simulink model "rfsoc4x2_ospfb_128"  (R2021a)
settings: Solver=VariableStepAuto  StartTime=0.0  StopTime=2048  RelTol=1e-3
undefined symbols (not defined in the file): pfb_coeff_gen_calc
libraries: xbsIndex_r4 x25898, casper_library_delays x113, casper_library_misc x68, xps_library x1
(part 1 of 221)
settings Model: Creator=leeke  LastModifiedBy=leeke

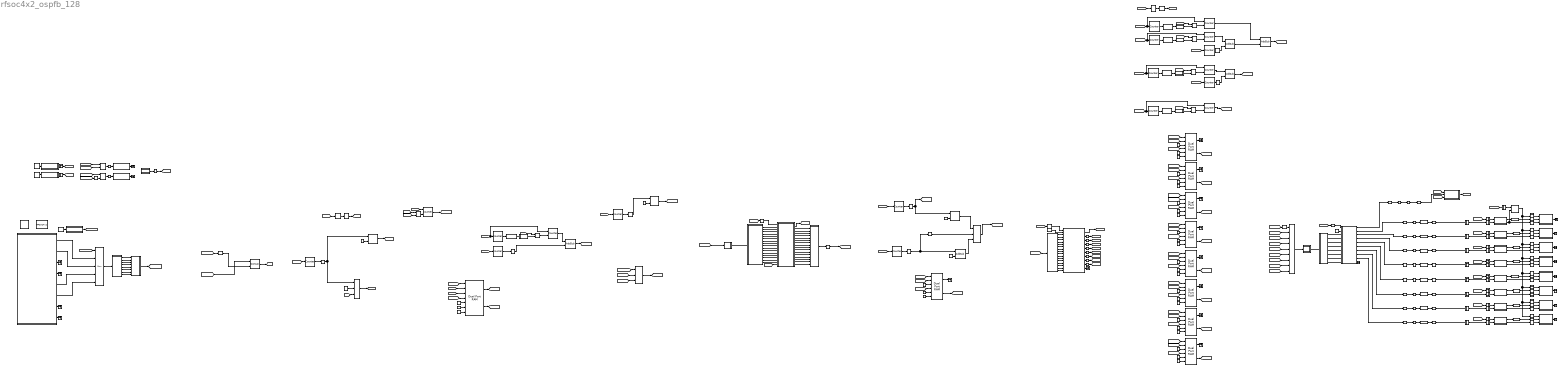
== system rfsoc4x2_ospfb_128 ==
  note: 2nd-stage channelizaton FFT
  note: Coner turn
  note: 1st-stage channelizaton OSPFB
  note: 2x Oversampled polyphase fiter banks
  note: 1st-stage channelizaton OSPFB > Corner Turn > 2nd-stage channelizaton FFT > output
  note: acc_cntrl has a clock
      | cycle latency in generating
      | new_acc signal.
      | Compensate by delaying
      | data here.
  note: 1delay RW mode
  " System Generator" : xbsIndex_r4/ System Generator  Tag=genX  xilinxfamily=zynquplusRFSOC  part=xczu48dr  speed=-2-e  package=ffvg1517  synthesis_tool=XST  clock_wrapper=Clock Enables  directory=/home/leeke/rfsoc4x2/leeke/project/burst/ospfb/2x/8/PFB_FFT/rfsoc4x2_ospfb_128/sysgen  proj_type=Vivado  Synth_file=Vivado Synthesis Defaults  Impl_file=Vivado Implementation Defaults  testbench=off  simulink_period=1  sysclk_period=5  dcm_input_clock_period=10  incr_netlist=off  trim_vbits=Everywhere in SubSystem  dbl_ovrd=According to Block Masks  core_generation=According to Block Masks  run_coregen=off  deprecated_control=off  eval_field=0  block_type=sysgen
  AddSub : xbsIndex_r4/AddSub  mode=Addition  use_carryin=off  use_carryout=off  en=off  latency=0  precision=User Defined  arith_type=Unsigned  n_bits=6-1  bin_pt=0  quantization=Truncate  overflow=Wrap  use_behavioral_HDL=off  hw_selection=Fabric  pipelined=off  dbl_ovrd=off  block_type=addsub
  AddSub1 : xbsIndex_r4/AddSub  mode=Addition  use_carryin=off  use_carryout=off  en=off  latency=0  precision=User Defined  arith_type=Unsigned  n_bits=15-1  bin_pt=0  quantization=Truncate  overflow=Wrap  use_behavioral_HDL=off  hw_selection=Fabric  pipelined=off  dbl_ovrd=off  block_type=addsub
  AddSub2 : xbsIndex_r4/AddSub  mode=Addition  use_carryin=off  use_carryout=off  en=off  latency=0  precision=User Defined  arith_type=Unsigned  n_bits=15-1  bin_pt=0  quantization=Truncate  overflow=Wrap  use_behavioral_HDL=off  hw_selection=Fabric  pipelined=off  dbl_ovrd=off  block_type=addsub
  AddSub3 : xbsIndex_r4/AddSub  mode=Addition  use_carryin=off  use_carryout=off  en=off  latency=0  precision=User Defined  arith_type=Unsigned  n_bits=11  bin_pt=0  quantization=Truncate  overflow=Wrap  use_behavioral_HDL=off  hw_selection=Fabric  pipelined=off  dbl_ovrd=off  block_type=addsub
  AddSub55 : xbsIndex_r4/AddSub  mode=Addition  use_carryin=off  use_carryout=off  en=off  latency=0  precision=User Defined  arith_type=Unsigned  n_bits=5-1  bin_pt=0  quantization=Truncate  overflow=Wrap  use_behavioral_HDL=off  hw_selection=Fabric  pipelined=off  dbl_ovrd=off  block_type=addsub
  Concat6 : xbsIndex_r4/Concat  num_inputs=2  dbl_ovrd=off  block_type=concat
  Constant : Constant  Value=0
  Constant1 : xbsIndex_r4/Constant  const=(2^8)-1  gui_display_data_type=Fixed-point  arith_type=Unsigned  n_bits=8  bin_pt=0  preci_type=Single  exp_width=8  frac_width=24  explicit_period=on  period=1  equ=P=C  opselect=C  inp2=PCIN>>17  opr=+  inp1=P  carry=CIN  dbl_ovrd=off  block_type=constant
  Constant{8..11,16,28,38,43,48} (9 alike) : xbsIndex_r4/Constant  const=1.0  gui_display_data_type=Boolean  arith_type=Boolean  n_bits=1  bin_pt=0  preci_type=Single  exp_width=8  frac_width=24  explicit_period=off  period=1  equ=P=C  opselect=C  inp2=PCIN>>17  opr=+  inp1=P  carry=CIN  dbl_ovrd=off  block_type=constant
  Constant109 : xbsIndex_r4/Constant  const=0  gui_display_data_type=Fixed-point  arith_type=Unsigned  n_bits=64  bin_pt=0  preci_type=Single  exp_width=8  frac_width=24  explicit_period=off  period=1  equ=P=C  opselect=C  inp2=PCIN>>17  opr=+  inp1=P  carry=CIN  dbl_ovrd=off  block_type=constant
  Constant110 : xbsIndex_r4/Constant  const=0  gui_display_data_type=Fixed-point  arith_type=Unsigned  n_bits=16 * 16  bin_pt=0  preci_type=Single  exp_width=8  frac_width=24  explicit_period=off  period=1  equ=P=C  opselect=C  inp2=PCIN>>17  opr=+  inp1=P  carry=CIN  dbl_ovrd=off  block_type=constant
  Constant{17,19,30,37,40,42,45,47,50,111} (10 alike) : xbsIndex_r4/Constant  const=0  gui_display_data_type=Boolean  arith_type=Boolean  n_bits=144  bin_pt=0  preci_type=Single  exp_width=8  frac_width=24  explicit_period=off  period=1  equ=P=C  opselect=C  inp2=PCIN>>17  opr=+  inp1=P  carry=CIN  dbl_ovrd=off  block_type=constant
  Constant112 : xbsIndex_r4/Constant  const=1  gui_display_data_type=Boolean  arith_type=Boolean  n_bits=144  bin_pt=0  preci_type=Single  exp_width=8  frac_width=24  explicit_period=off  period=1  equ=P=C  opselect=C  inp2=PCIN>>17  opr=+  inp1=P  carry=CIN  dbl_ovrd=off  block_type=constant
  Constant113 : xbsIndex_r4/Constant  const=0  gui_display_data_type=Fixed-point  arith_type=Unsigned  n_bits=1  bin_pt=0  preci_type=Single  exp_width=8  frac_width=24  explicit_period=off  period=1  equ=P=C  opselect=C  inp2=PCIN>>17  opr=+  inp1=P  carry=CIN  dbl_ovrd=off  block_type=constant
  Constant114 : xbsIndex_r4/Constant  const=(2^8 / 2^4) - 1  gui_display_data_type=Fixed-point  arith_type=Unsigned  n_bits=log2((2^8 / 2^4))  bin_pt=0  preci_type=Single  exp_width=8  frac_width=24  explicit_period=off  period=1  equ=P=C  opselect=C  inp2=PCIN>>17  opr=+  inp1=P  carry=CIN  dbl_ovrd=off  block_type=constant
  Constant{12..13,18,29,39,41,44,46,49} (9 alike) : xbsIndex_r4/Constant  const=0  gui_display_data_type=Fixed-point  arith_type=Unsigned  n_bits=144*2  bin_pt=0  preci_type=Single  exp_width=8  frac_width=24  explicit_period=off  period=1  equ=P=C  opselect=C  inp2=PCIN>>17  opr=+  inp1=P  carry=CIN  dbl_ovrd=off  block_type=constant
  Constant2 : Constant  Value=0
  Constant20 : xbsIndex_r4/Constant  const=32/2  gui_display_data_type=Fixed-point  arith_type=Unsigned  n_bits=6-1  bin_pt=0  preci_type=Single  exp_width=8  frac_width=24  explicit_period=off  period=1  equ=P=C  opselect=C  inp2=PCIN>>17  opr=+  inp1=P  carry=CIN  dbl_ovrd=off  block_type=constant
  Constant21 : xbsIndex_r4/Constant  const=32/2  gui_display_data_type=Fixed-point  arith_type=Unsigned  n_bits=6-1  bin_pt=0  preci_type=Single  exp_width=8  frac_width=24  explicit_period=off  period=1  equ=P=C  opselect=C  inp2=PCIN>>17  opr=+  inp1=P  carry=CIN  dbl_ovrd=off  block_type=constant
  Constant3 : Constant  Value=2
  Constant51 : xbsIndex_r4/Constant  const=(2^9)-1  gui_display_data_type=Fixed-point  arith_type=Unsigned  n_bits=9  bin_pt=0  preci_type=Single  exp_width=8  frac_width=24  explicit_period=on  period=1  equ=P=C  opselect=C  inp2=PCIN>>17  opr=+  inp1=P  carry=CIN  dbl_ovrd=off  block_type=constant
  Convert2 : xbsIndex_r4/Convert  gui_display_data_type=Boolean  arith_type=Boolean  n_bits=16  bin_pt=14  float_type=Single  exp_bits=8  fraction_bits=24  quantization=Truncate  overflow=Wrap  en=off  latency=1  pipeline=off  dbl_ovrd=off  block_type=convert
  Convert6 : xbsIndex_r4/Convert  gui_display_data_type=Boolean  arith_type=Boolean  n_bits=16  bin_pt=14  float_type=Single  exp_bits=8  fraction_bits=24  quantization=Truncate  overflow=Wrap  en=off  latency=1  pipeline=off  dbl_ovrd=off  block_type=convert
  Counter1 : xbsIndex_r4/Counter  cnt_type=Count Limited  cnt_to=(16384/2)-512  operation=Up  start_count=0  cnt_by_val=512  arith_type=Unsigned  n_bits=14-1  bin_pt=0  load_pin=off  rst=on  en=off  explicit_period=on  period=1  use_behavioral_HDL=off  implementation=Fabric  dbl_ovrd=off  block_type=counter
  Counter13 : xbsIndex_r4/Counter  cnt_type=Free Running  cnt_to=1023  operation=Up  start_count=16/2  cnt_by_val=1  arith_type=Unsigned  n_bits=5-1  bin_pt=0  load_pin=off  rst=on  en=off  explicit_period=on  period=1  use_behavioral_HDL=off  implementation=Fabric  dbl_ovrd=off  block_type=counter
  Counter14 : xbsIndex_r4/Counter  cnt_type=Free Running  cnt_to=Inf  operation=Up  start_count=0  cnt_by_val=1  arith_type=Unsigned  n_bits=7-1  bin_pt=0  load_pin=off  rst=on  en=off  explicit_period=on  period=1  use_behavioral_HDL=off  implementation=Fabric  dbl_ovrd=off  block_type=counter
  Counter15 : xbsIndex_r4/Counter  cnt_type=Free Running  cnt_to=1023  operation=Up  start_count=0  cnt_by_val=1  arith_type=Unsigned  n_bits=6-1  bin_pt=0  load_pin=off  rst=on  en=off  explicit_period=on  period=1  use_behavioral_HDL=off  implementation=Fabric  dbl_ovrd=off  block_type=counter
  Counter16 : xbsIndex_r4/Counter  cnt_type=Free Running  cnt_to=Inf  operation=Up  start_count=0  cnt_by_val=1  arith_type=Unsigned  n_bits=7-1  bin_pt=0  load_pin=off  rst=on  en=off  explicit_period=on  period=1  use_behavioral_HDL=off  implementation=Fabric  dbl_ovrd=off  block_type=counter
  Counter17 : xbsIndex_r4/Counter  cnt_type=Free Running  cnt_to=16  operation=Up  start_count=1024  cnt_by_val=128/2  arith_type=Unsigned  n_bits=11  bin_pt=0  load_pin=off  rst=on  en=on  explicit_period=on  period=1  use_behavioral_HDL=off  implementation=Fabric  dbl_ovrd=off  block_type=counter
  Counter18 : xbsIndex_r4/Counter  cnt_type=Free Running  cnt_to=Inf  operation=Up  start_count=0  cnt_by_val=1  arith_type=Unsigned  n_bits=9  bin_pt=0  load_pin=off  rst=on  en=off  explicit_period=on  period=1  use_behavioral_HDL=off  implementation=Fabric  dbl_ovrd=off  block_type=counter
  Counter19 : xbsIndex_r4/Counter  cnt_type=Free Running  cnt_to=Inf  operation=Up  start_count=0  cnt_by_val=1  arith_type=Unsigned  n_bits=1  bin_pt=0  load_pin=off  rst=off  en=on  explicit_period=on  period=1  use_behavioral_HDL=off  implementation=Fabric  dbl_ovrd=off  block_type=counter
  Counter2 : xbsIndex_r4/Counter  cnt_type=Free Running  cnt_to=0  operation=Up  start_count=0  cnt_by_val=1  arith_type=Unsigned  n_bits=9  bin_pt=0  load_pin=off  rst=on  en=on  explicit_period=on  period=1  use_behavioral_HDL=off  implementation=Fabric  dbl_ovrd=off  block_type=counter
  Counter3 : xbsIndex_r4/Counter  cnt_type=Free Running  cnt_to=0  operation=Up  start_count=0  cnt_by_val=16384/2  arith_type=Unsigned  n_bits=15-1  bin_pt=0  load_pin=off  rst=on  en=on  explicit_period=on  period=1  use_behavioral_HDL=off  implementation=Fabric  dbl_ovrd=off  block_type=counter
  Counter4 : xbsIndex_r4/Counter  cnt_type=Free Running  cnt_to=Inf  operation=Up  start_count=0  cnt_by_val=1  arith_type=Unsigned  n_bits=14-1  bin_pt=0  load_pin=off  rst=on  en=off  explicit_period=on  period=1  use_behavioral_HDL=off  implementation=Fabric  dbl_ovrd=off  block_type=counter
  Counter55 : xbsIndex_r4/Counter  cnt_type=Free Running  cnt_to=1023  operation=Up  start_count=0  cnt_by_val=1  arith_type=Unsigned  n_bits=1  bin_pt=0  load_pin=off  rst=on  en=off  explicit_period=on  period=1  use_behavioral_HDL=off  implementation=Fabric  dbl_ovrd=off  block_type=counter
  Counter56 : xbsIndex_r4/Counter  cnt_type=Free Running  cnt_to=1023  operation=Up  start_count=0  cnt_by_val=1  arith_type=Unsigned  n_bits=log2((2^8 / 2^4))  bin_pt=0  load_pin=off  rst=on  en=on  explicit_period=on  period=1  use_behavioral_HDL=off  implementation=Fabric  dbl_ovrd=off  block_type=counter
  Counter57 : xbsIndex_r4/Counter  cnt_type=Free Running  cnt_to=Inf  operation=Up  start_count=0  cnt_by_val=1  arith_type=Unsigned  n_bits=1  bin_pt=0  load_pin=off  rst=off  en=on  explicit_period=on  period=1  use_behavioral_HDL=off  implementation=Fabric  dbl_ovrd=off  block_type=counter
  Counter58 : xbsIndex_r4/Counter  cnt_type=Free Running  cnt_to=0  operation=Up  start_count=8  cnt_by_val=16/2  arith_type=Unsigned  n_bits=5-1  bin_pt=0  load_pin=off  rst=on  en=on  explicit_period=on  period=1  use_behavioral_HDL=off  implementation=Fabric  dbl_ovrd=off  block_type=counter
  Counter59 : xbsIndex_r4/Counter  cnt_type=Free Running  cnt_to=Inf  operation=Up  start_count=16/2  cnt_by_val=1  arith_type=Unsigned  n_bits=5-1  bin_pt=0  load_pin=off  rst=on  en=off  explicit_period=on  period=1  use_behavioral_HDL=off  implementation=Fabric  dbl_ovrd=off  block_type=counter
  Counter6 : xbsIndex_r4/Counter  cnt_type=Free Running  cnt_to=Inf  operation=Up  start_count=0  cnt_by_val=1  arith_type=Unsigned  n_bits=5-1  bin_pt=0  load_pin=off  rst=on  en=off  explicit_period=on  period=1  use_behavioral_HDL=off  implementation=Fabric  dbl_ovrd=off  block_type=counter
  Counter60 : xbsIndex_r4/Counter  cnt_type=Free Running  cnt_to=1023  operation=Up  start_count=0  cnt_by_val=1  arith_type=Unsigned  n_bits=4-1  bin_pt=0  load_pin=off  rst=on  en=off  explicit_period=on  period=1  use_behavioral_HDL=off  implementation=Fabric  dbl_ovrd=off  block_type=counter
  Counter61 : xbsIndex_r4/Counter  cnt_type=Free Running  cnt_to=1023  operation=Up  start_count=0  cnt_by_val=1  arith_type=Unsigned  n_bits=log2((2^8 / 2^4))  bin_pt=0  load_pin=off  rst=on  en=off  explicit_period=on  period=1  use_behavioral_HDL=off  implementation=Fabric  dbl_ovrd=off  block_type=counter
  Counter7 : xbsIndex_r4/Counter  cnt_type=Free Running  cnt_to=16  operation=Up  start_count=0  cnt_by_val=1  arith_type=Unsigned  n_bits=2+1  bin_pt=0  load_pin=off  rst=on  en=on  explicit_period=on  period=1  use_behavioral_HDL=off  implementation=Fabric  dbl_ovrd=off  block_type=counter
  Delay{1..4,49..50,57..58,62,66,68..71,74..75,77..78,81,83..87,89..90} (26 alike) : xbsIndex_r4/Delay  rst=off  infoeditControl=Selection of Reset will increase slice count due to use of real FFs and instead of SRLs  en=off  latency=1  reg_retiming=on  dbl_ovrd=off  block_type=delay
  Delay{13..14,17,23,59..61,136..139} (11 alike) : xbsIndex_r4/Delay  rst=off  infoeditControl=Selection of Reset will increase slice count due to use of real FFs and instead of SRLs  en=off  latency=1  reg_retiming=off  dbl_ovrd=off  block_type=delay
  Delay15 : xbsIndex_r4/Delay  rst=off  infoeditControl=Selection of Reset will increase slice count due to use of real FFs and instead of SRLs  en=off  latency=16/2  reg_retiming=off  dbl_ovrd=off  block_type=delay
  Delay16 : xbsIndex_r4/Delay  rst=off  infoeditControl=Selection of Reset will increase slice count due to use of real FFs and instead of SRLs  en=off  latency=2  reg_retiming=off  dbl_ovrd=off  block_type=delay
  Delay{6,21,33,63..65,67,72,76,79..80,82,88} (13 alike) : xbsIndex_r4/Delay  rst=off  infoeditControl=Selection of Reset will increase slice count due to use of real FFs and instead of SRLs  en=off  latency=2  reg_retiming=on  dbl_ovrd=off  block_type=delay
  Delay73 : xbsIndex_r4/Delay  rst=off  infoeditControl=Selection of Reset will increase slice count due to use of real FFs and instead of SRLs  en=off  latency=5  reg_retiming=on  dbl_ovrd=off  block_type=delay
  Dual Port RAM{1..4,11..14} (8 alike) : xbsIndex_r4/Dual Port RAM  depth=16384  initVector=0  distributed_mem=Block RAM  init_a=0  init_b=0  rst_a=off  rst_b=off  en_a=off  en_b=off  latency=1  write_mode_A=Read Before Write  write_mode_B=Read Before Write  optimize=Area  dbl_ovrd=off  simulation_type=fast_sim  block_type=dpram
  Dual Port RAM16 : xbsIndex_r4/Dual Port RAM  depth=(2^8) / (2^4)  initVector=0  distributed_mem=Block RAM  init_a=0  init_b=0  rst_a=off  rst_b=off  en_a=off  en_b=on  latency=1  write_mode_A=Read After Write  write_mode_B=Read Before Write  optimize=Area  dbl_ovrd=off  simulation_type=fast_sim  block_type=dpram
  Dual Port RAM6 : xbsIndex_r4/Dual Port RAM  depth=32  initVector=0  distributed_mem=Block RAM  init_a=0  init_b=0  rst_a=off  rst_b=off  en_a=off  en_b=off  latency=1  write_mode_A=Read Before Write  write_mode_B=Read Before Write  optimize=Area  dbl_ovrd=off  simulation_type=fast_sim  block_type=dpram
  Logical{2..3,9..10,12..13} (6 alike) : xbsIndex_r4/Logical  logical_function=AND  inputs=2  en=off  latency=0  precision=Full  arith_type=Unsigned  n_bits=16  bin_pt=0  align_bp=on  dbl_ovrd=off  block_type=logical
  Mux : xbsIndex_r4/Mux  inputs=4  en=off  latency=2  precision=Full  arith_type=Unsigned  n_bits=16  bin_pt=14  quantization=Truncate  overflow=Wrap  dbl_ovrd=off  block_type=mux
  Mux13 : xbsIndex_r4/Mux  inputs=2  en=off  latency=0  precision=Full  arith_type=Unsigned  n_bits=16  bin_pt=14  quantization=Truncate  overflow=Wrap  dbl_ovrd=off  block_type=mux
  Mux14 : xbsIndex_r4/Mux  inputs=2  en=off  latency=0  precision=Full  arith_type=Unsigned  n_bits=16  bin_pt=14  quantization=Truncate  overflow=Wrap  dbl_ovrd=off  block_type=mux
  Mux3 : xbsIndex_r4/Mux  inputs=2  en=off  latency=0  precision=Full  arith_type=Unsigned  n_bits=16  bin_pt=14  quantization=Truncate  overflow=Wrap  dbl_ovrd=off  block_type=mux
  Mux5 : xbsIndex_r4/Mux  inputs=8  en=off  latency=0  precision=Full  arith_type=Unsigned  n_bits=16  bin_pt=14  quantization=Truncate  overflow=Wrap  dbl_ovrd=off  block_type=mux
  RFSoC4x2 : xps_library/Platforms/RFSoC4x2  Tag=xps:xsg  hw_sys=rfsoc4x2:xczu48dr  clk_src=adc_clk  clk_rate=200  pl_clk_rate=100  sample_period=1  synthesis_tool=XST
      settings: SourceProductName=CASPER XPS Blockset
  Reinterpret{7,10..16} (8 alike) : xbsIndex_r4/Reinterpret  force_arith_type=on  arith_type=Unsigned  force_bin_pt=on  bin_pt=0  block_type=reinterpret
      settings: infoedit="Changes signal type without altering the binary representation.   You can changed the signal between signed and unsigned, and relocate the binary point.<P><P>Hardware notes: In hardware this block costs nothing.<P><P>Example:  Suppose the input is 6 bits wide, signed, with 2 fractional bits, and the output is forced to unsigned with 0 fractional bits.  Then an input of -2.0 (1110.00 in binary 2's complement) becomes an output of 56 (111000 in binary)."  block_version=10.1.3
  Relational : xbsIndex_r4/Relational  mode=a<b  op_type=Bool  en=off  latency=0  dbl_ovrd=off  block_type=relational
  Relational2 : xbsIndex_r4/Relational  mode=a>b  op_type=Bool  en=off  latency=0  dbl_ovrd=off  block_type=relational
  Relational3 : xbsIndex_r4/Relational  mode=a<b  op_type=Bool  en=off  latency=1  dbl_ovrd=off  block_type=relational
  Slice{1,3..5,14} (5 alike) : xbsIndex_r4/Slice  nbits=1  boolean_output=on  mode=Upper Bit Location + Width  bit1=0  base1=MSB of Input  bit0=0  base0=LSB of Input  dbl_ovrd=off  block_type=slice
  Terminator{1..4,6..7,11,16,18..23,25..34,38} (25 alike) : Terminator
  acc_cnt : Subsystem  Tag=xps:sw_reg  AncestorBlock=xps_library/Memory/software_register  mask(swreg){io_dir=To Processor, io_delay=0, init_val=0, sample_period=1, names=reg, bitwidths=32, bin_pts=0, arith_types=0, sim_port=on, show_format=off}
      mask prompts: io_dir "I/O direction"; io_delay "I/O delay"; init_val "Initial Value"; sample_period "Sample period"; names "Bitfield names [msb...lsb]"; bitwidths "Bitfield widths"; bin_pts "Bitfield binary pts"; arith_types "Bitfield types, ufix=0, fix=1, bool=2"; sim_port "Provide sim input/output?"; show_format "Print format string?"
      mask help: A 32-bit software-accessible register. Can be divided into bitfields of varying widths and types using the fields in the block mask.
      mask init:
      | swreg_init(gcb)
      settings: AttributesFormatString=1output
      mask TypeOptions io_dir: To Processor | From Processor
      mask Callback io_dir:
      | mask_enables = get_param(gcb, 'MaskEnables');
      | mask_names = get_param(gcb, 'MaskNames');
      | if strcmp(get_param(gcb, 'io_dir'), 'To Processor'),
      |     mask_enables{ismember(mask_names, 'sample_period')} = 'off';
      | else
      |     mask_enables{ismember(mask_names, 'sample_period')} = 'on';
      | end
      | set_param(gcb, 'MaskEnables', mask_enables);
      mask DialogControl ParameterTabVar0 Prompt: Setup
  acc_cntr : xbsIndex_r4/Counter  cnt_type=Free Running  cnt_to=Inf  operation=Up  start_count=0  cnt_by_val=1  arith_type=Unsigned  n_bits=32  bin_pt=0  load_pin=off  rst=on  en=on  explicit_period=on  period=1  use_behavioral_HDL=off  implementation=Fabric  use_rpm=off  dbl_ovrd=off  block_type=counter
  acc_cntrl2 : Subsystem  mask{chan_bits=13}
      mask prompts: chan_bits "Number of Channels (2^?)"
  acc_len : Subsystem  Tag=xps:sw_reg  AncestorBlock=xps_library/Memory/software_register  mask(swreg){io_dir=From Processor, io_delay=0, init_val=0, sample_period=1, names=reg, bitwidths=32, bin_pts=0, arith_types=0, sim_port=on, show_format=off}
      mask prompts: io_dir "I/O direction"; io_delay "I/O delay"; init_val "Initial Value"; sample_period "Sample period"; names "Bitfield names [msb...lsb]"; bitwidths "Bitfield widths"; bin_pts "Bitfield binary pts"; arith_types "Bitfield types, ufix=0, fix=1, bool=2"; sim_port "Provide sim input/output?"; show_format "Print format string?"
      mask help: A 32-bit software-accessible register. Can be divided into bitfields of varying widths and types using the fields in the block mask.
      mask init:
      | swreg_init(gcb)
      settings: AttributesFormatString=1input
      mask TypeOptions io_dir: To Processor | From Processor
      mask Callback io_dir:
      | mask_enables = get_param(gcb, 'MaskEnables');
      | mask_names = get_param(gcb, 'MaskNames');
      | if strcmp(get_param(gcb, 'io_dir'), 'To Processor'),
      |     mask_enables{ismember(mask_names, 'sample_period')} = 'off';
      | else
      |     mask_enables{ismember(mask_names, 'sample_period')} = 'on';
      | end
      | set_param(gcb, 'MaskEnables', mask_enables);
      mask DialogControl ParameterTabVar0 Prompt: Setup
  adc_chan_sel : Subsystem  Tag=xps:sw_reg  AncestorBlock=xps_library/Memory/software_register  mask(swreg){io_dir=From Processor, io_delay=0, init_val=dec2hex(0), sample_period=1, names=reg, bitwidths=2, bin_pts=0, arith_types=0, sim_port=on, show_format=on}
      mask prompts: io_dir "I/O direction"; io_delay "I/O delay"; init_val "Initial Value"; sample_period "Sample period"; names "Bitfield names [msb...lsb]"; bitwidths "Bitfield widths"; bin_pts "Bitfield binary pts"; arith_types "Bitfield types, ufix=0, fix=1, bool=2"; sim_port "Provide sim input/output?"; show_format "Print format string?"
      mask help: A 32-bit software-accessible register. Can be divided into bitfields of varying widths and types using the fields in the block mask.
      mask init:
      | swreg_init(gcb)
      settings: AttributesFormatString=1input:uf2.0 = 2 bits
      mask TypeOptions io_dir: To Processor | From Processor
      mask Callback io_dir:
      | mask_enables = get_param(gcb, 'MaskEnables');
      | mask_names = get_param(gcb, 'MaskNames');
      | if strcmp(get_param(gcb, 'io_dir'), 'To Processor'),
      |     mask_enables{ismember(mask_names, 'sample_period')} = 'off';
      | else
      |     mask_enables{ismember(mask_names, 'sample_period')} = 'on';
      | end
      | set_param(gcb, 'MaskEnables', mask_enables);
      mask DialogControl ParameterTabVar0 Prompt: Setup
  bus_create : Subsystem  AncestorBlock=casper_library_flow_control/bus_create  mask(bus_create){inputNum=8}
      mask prompts: inputNum "Number of inputs:"
      mask init:
      | bus_create_init(gcb,...
      |     'inputNum', inputNum);
  bus_create2 : Subsystem  AncestorBlock=casper_library_flow_control/bus_create  mask(bus_create){inputNum=16}
      mask prompts: inputNum "Number of inputs:"
      mask init:
      | bus_create_init(gcb,...
      |     'inputNum', inputNum);
  bus_expand : Subsystem  AncestorBlock=casper_library_flow_control/bus_expand  mask(bus_expand){mode=divisions of equal size, outputNum=16, outputWidth=16, outputBinaryPt=0, outputArithmeticType=0, show_format=off, outputToWorkspace=off, variablePrefix=out, outputToModelAsWell=on}
      mask prompts: outputNum "Number of outputs:"; outputWidth "Output width:"; outputBinaryPt "Output binary point position:"; outputArithmeticType "Output arithmetic type (ufix=0, fix=1, bool=2):"; show_format "Print format string?"; outputToWorkspace "Output to workspace?"; variablePrefix "Variable name prefix:"; outputToModelAsWell "Output to model as well?"
      mask help:
      | Expands a 'bus' made using a bus_create or Xilinx
      | concat block.
      | The input will be divided into the specified number
      | of outputs with the specified arithmetic types.
      | Divisions are made from most significant bit.
      mask init:
      | bus_expand_init(gcb,...
      |     'mode', mode, ...
      |     'outputNum', outputNum, ...
      |     'outputWidth', outputWidth, ...
      |     'outputBinaryPt', outputBinaryPt, ...
      |     'outputArithmeticType', outputArithmeticType, ...
      |     'show_format', show_format, ...
      |     'outputToWorkspace', outputToWorkspace, ...
      |     'variablePrefix', variablePrefix, ...
      |     'outputToModelAsWell', outputToModelAsWell);
      settings: AttributesFormatString=16 outputs
      mask TypeOptions mode: divisions of equal size | divisions of arbitrary size
      mask Callback mode: %bus_expand_callback();
      mask Callback outputWidth: %bus_expand_callback();
      mask Callback outputToWorkspace: %bus_expand_callback();
  bus_expand1 : Subsystem  AncestorBlock=casper_library_flow_control/bus_expand  mask(bus_expand){mode=divisions of equal size, outputNum=8, outputWidth=16, outputBinaryPt=0, outputArithmeticType=0, show_format=off, outputToWorkspace=off, variablePrefix=out, outputToModelAsWell=on}
      mask prompts: outputNum "Number of outputs:"; outputWidth "Output width:"; outputBinaryPt "Output binary point position:"; outputArithmeticType "Output arithmetic type (ufix=0, fix=1, bool=2):"; show_format "Print format string?"; outputToWorkspace "Output to workspace?"; variablePrefix "Variable name prefix:"; outputToModelAsWell "Output to model as well?"
      mask help:
      | Expands a 'bus' made using a bus_create or Xilinx
      | concat block.
      | The input will be divided into the specified number
      | of outputs with the specified arithmetic types.
      | Divisions are made from most significant bit.
      mask init: same as rfsoc4x2_ospfb_128/bus_expand
      settings: AttributesFormatString=8 outputs
      mask TypeOptions mode: divisions of equal size | divisions of arbitrary size
      mask Callback mode: %bus_expand_callback();
      mask Callback outputWidth: %bus_expand_callback();
      mask Callback outputToWorkspace: %bus_expand_callback();
  bus_expand3 : Subsystem  AncestorBlock=casper_library_flow_control/bus_expand  mask(bus_expand){mode=divisions of equal size, outputNum=16, outputWidth=18, outputBinaryPt=17, outputArithmeticType=1, show_format=off, outputToWorkspace=off, variablePrefix=out, outputToModelAsWell=on}
      mask prompts: outputNum "Number of outputs:"; outputWidth "Output width:"; outputBinaryPt "Output binary point position:"; outputArithmeticType "Output arithmetic type (ufix=0, fix=1, bool=2):"; show_format "Print format string?"; outputToWorkspace "Output to workspace?"; variablePrefix "Variable name prefix:"; outputToModelAsWell "Output to model as well?"
      mask help:
      | Expands a 'bus' made using a bus_create or Xilinx
      | concat block.
      | The input will be divided into the specified number
      | of outputs with the specified arithmetic types.
      | Divisions are made from most significant bit.
      mask init: same as rfsoc4x2_ospfb_128/bus_expand
      settings: AttributesFormatString=16 outputs
      mask TypeOptions mode: divisions of equal size | divisions of arbitrary size
      mask Callback mode: %bus_expand_callback();
      mask Callback outputWidth: %bus_expand_callback();
      mask Callback outputToWorkspace: %bus_expand_callback();
  bus_expand4 : Subsystem  AncestorBlock=casper_library_flow_control/bus_expand  mask(bus_expand){mode=divisions of equal size, outputNum=8, outputWidth=36, outputBinaryPt=0, outputArithmeticType=0, show_format=off, outputToWorkspace=off, variablePrefix=out, outputToModelAsWell=on}
      mask prompts: outputNum "Number of outputs:"; outputWidth "Output width:"; outputBinaryPt "Output binary point position:"; outputArithmeticType "Output arithmetic type (ufix=0, fix=1, bool=2):"; show_format "Print format string?"; outputToWorkspace "Output to workspace?"; variablePrefix "Variable name prefix:"; outputToModelAsWell "Output to model as well?"
      mask help:
      | Expands a 'bus' made using a bus_create or Xilinx
      | concat block.
      | The input will be divided into the specified number
      | of outputs with the specified arithmetic types.
      | Divisions are made from most significant bit.
      mask init: same as rfsoc4x2_ospfb_128/bus_expand
      settings: AttributesFormatString=8 outputs
      mask TypeOptions mode: divisions of equal size | divisions of arbitrary size
      mask Callback mode: %bus_expand_callback();
      mask Callback outputWidth: %bus_expand_callback();
      mask Callback outputToWorkspace: %bus_expand_callback();
  cnt_rst : Subsystem  Tag=xps:sw_reg  AncestorBlock=xps_library/Memory/software_register  mask(swreg){io_dir=From Processor, io_delay=0, init_val=dec2hex(0), sample_period=1, names=reg, bitwidths=1, bin_pts=0, arith_types=2, sim_port=on, show_format=on}
      mask prompts: io_dir "I/O direction"; io_delay "I/O delay"; init_val "Initial Value"; sample_period "Sample period"; names "Bitfield names [msb...lsb]"; bitwidths "Bitfield widths"; bin_pts "Bitfield binary pts"; arith_types "Bitfield types, ufix=0, fix=1, bool=2"; sim_port "Provide sim input/output?"; show_format "Print format string?"
      mask help: A 32-bit software-accessible register. Can be divided into bitfields of varying widths and types using the fields in the block mask.
      mask init:
      | swreg_init(gcb)
      settings: AttributesFormatString=1input:b = 1 bits
      mask TypeOptions io_dir: To Processor | From Processor
      mask Callback io_dir:
      | mask_enables = get_param(gcb, 'MaskEnables');
      | mask_names = get_param(gcb, 'MaskNames');
      | if strcmp(get_param(gcb, 'io_dir'), 'To Processor'),
      |     mask_enables{ismember(mask_names, 'sample_period')} = 'off';
      | else
      |     mask_enables{ismember(mask_names, 'sample_period')} = 'on';
      | end
      | set_param(gcb, 'MaskEnables', mask_enables);
      mask DialogControl ParameterTabVar0 Prompt: Setup
  edge_detect1 : Subsystem  AncestorBlock=casper_library_misc/edge_detect  mask(edge_detect){edge=Falling, polarity=Active High, x_in=[0 0.08 0.08 0.16 0.16 0.24 0.24 0.32 0.32 0.4], y_in=[-1 -1  1  1  1  1  1  1  1  1], x_out=[0.6 0.68 0.68 0.76 0.76 0.84 0.84 0.92 0.92 1], y_out=[-1 -1  1  1 -1 -1 -1 -1 -1 -1]}
      mask prompts: edge "Edge Type"; polarity "Output Polarity"; x_in "Input X Positions"; y_in "Input Y Positions"; x_out "Output X Positions"; y_out "Output Y Positions"
      mask help: Output is active for one-cycle after each edge of the specified type (i.e. rising, falling or both).
      mask init:
      | edge_detect_init(gcb,...
      |     'edge',edge,...
      |     'polarity',polarity,...
      |     'x_in',x_in,...
      |     'x_out',x_out,...
      |     'y_in',y_in,...
      |     'y_out',y_out);
      | 
      | x_in_num=str2num(getfield(getfield(get_param(gcb,'UserData'),'parameters'),'x_in'));
      | x_out_num=str2num(getfield(getfield(get_param(gcb,'UserData'),'parameters'),'x_out'));
      | y_in_num=str2num(getfield(getfield(get_param(gcb,'UserData'),'parameters'),'y_in'));
      | y_out_num=str2num(getfield(getfield(get_param(gcb,'UserData'),'parameters'),'y_out'));
      settings: AttributesFormatString=|
      | falling edges
      | active high
      mask Help: Output is active for one-cycle after each edge of the specified type (i.e. rising, falling, or both).  Latency is zero.
      mask TypeOptions edge: Rising | Falling | Both
      mask TypeOptions polarity: Active High | Active Low
      mask Display:
      | plot(x_in_num,0.5+y_in_num*0.2);
      | plot(x_out_num,0.5+y_out_num*0.2);
  edge_detect15 : Subsystem  AncestorBlock=casper_library_misc/edge_detect  mask(edge_detect){edge=Falling, polarity=Active High, x_in=[0 0.08 0.08 0.16 0.16 0.24 0.24 0.32 0.32 0.4], y_in=[-1 -1  1  1  1  1  1  1  1  1], x_out=[0.6 0.68 0.68 0.76 0.76 0.84 0.84 0.92 0.92 1], y_out=[-1 -1  1  1 -1 -1 -1 -1 -1 -1]}
      mask prompts: edge "Edge Type"; polarity "Output Polarity"; x_in "Input X Positions"; y_in "Input Y Positions"; x_out "Output X Positions"; y_out "Output Y Positions"
      mask help: Output is active for one-cycle after each edge of the specified type (i.e. rising, falling or both).
      mask init: same as rfsoc4x2_ospfb_128/edge_detect1
      settings: AttributesFormatString=|
      | falling edges
      | active high
      mask Help: Output is active for one-cycle after each edge of the specified type (i.e. rising, falling, or both).  Latency is zero.
      mask TypeOptions edge: Rising | Falling | Both
      mask TypeOptions polarity: Active High | Active Low
      mask Display:
      | plot(x_in_num,0.5+y_in_num*0.2);
      | plot(x_out_num,0.5+y_out_num*0.2);
  edge_detect2 : Subsystem  AncestorBlock=casper_library_misc/edge_detect  mask(edge_detect){edge=Falling, polarity=Active High, x_in=[0 0.08 0.08 0.16 0.16 0.24 0.24 0.32 0.32 0.4], y_in=[-1 -1  1  1  1  1  1  1  1  1], x_out=[0.6 0.68 0.68 0.76 0.76 0.84 0.84 0.92 0.92 1], y_out=[-1 -1  1  1 -1 -1 -1 -1 -1 -1]}
      mask prompts: edge "Edge Type"; polarity "Output Polarity"; x_in "Input X Positions"; y_in "Input Y Positions"; x_out "Output X Positions"; y_out "Output Y Positions"
      mask help: Output is active for one-cycle after each edge of the specified type (i.e. rising, falling or both).
      mask init: same as rfsoc4x2_ospfb_128/edge_detect1
      settings: AttributesFormatString=|
      | falling edges
      | active high
      mask Help: Output is active for one-cycle after each edge of the specified type (i.e. rising, falling, or both).  Latency is zero.
      mask TypeOptions edge: Rising | Falling | Both
      mask TypeOptions polarity: Active High | Active Low
      mask Display:
      | plot(x_in_num,0.5+y_in_num*0.2);
      | plot(x_out_num,0.5+y_out_num*0.2);
  edge_detect3 : Subsystem  AncestorBlock=casper_library_misc/edge_detect  mask(edge_detect){edge=Falling, polarity=Active High, x_in=[0 0.08 0.08 0.16 0.16 0.24 0.24 0.32 0.32 0.4], y_in=[-1 -1  1  1  1  1  1  1  1  1], x_out=[0.6 0.68 0.68 0.76 0.76 0.84 0.84 0.92 0.92 1], y_out=[-1 -1  1  1 -1 -1 -1 -1 -1 -1]}
      mask prompts: edge "Edge Type"; polarity "Output Polarity"; x_in "Input X Positions"; y_in "Input Y Positions"; x_out "Output X Positions"; y_out "Output Y Positions"
      mask help: Output is active for one-cycle after each edge of the specified type (i.e. rising, falling or both).
      mask init: same as rfsoc4x2_ospfb_128/edge_detect1
      settings: AttributesFormatString=|
      | falling edges
      | active high
      mask Help: Output is active for one-cycle after each edge of the specified type (i.e. rising, falling, or both).  Latency is zero.
      mask TypeOptions edge: Rising | Falling | Both
      mask TypeOptions polarity: Active High | Active Low
      mask Display:
      | plot(x_in_num,0.5+y_in_num*0.2);
      | plot(x_out_num,0.5+y_out_num*0.2);
  edge_detect4 : Subsystem  AncestorBlock=casper_library_misc/edge_detect  mask(edge_detect){edge=Falling, polarity=Active High, x_in=[0 0.08 0.08 0.16 0.16 0.24 0.24 0.32 0.32 0.4], y_in=[-1 -1  1  1  1  1  1  1  1  1], x_out=[0.6 0.68 0.68 0.76 0.76 0.84 0.84 0.92 0.92 1], y_out=[-1 -1  1  1 -1 -1 -1 -1 -1 -1]}
      mask prompts: edge "Edge Type"; polarity "Output Polarity"; x_in "Input X Positions"; y_in "Input Y Positions"; x_out "Output X Positions"; y_out "Output Y Positions"
      mask help: Output is active for one-cycle after each edge of the specified type (i.e. rising, falling or both).
      mask init: same as rfsoc4x2_ospfb_128/edge_detect1
      settings: AttributesFormatString=|
      | falling edges
      | active high
      mask Help: Output is active for one-cycle after each edge of the specified type (i.e. rising, falling, or both).  Latency is zero.
      mask TypeOptions edge: Rising | Falling | Both
      mask TypeOptions polarity: Active High | Active Low
      mask Display:
      | plot(x_in_num,0.5+y_in_num*0.2);
      | plot(x_out_num,0.5+y_out_num*0.2);
  fft1 : Subsystem  Tag=casper:fft  AncestorBlock=casper_library_ffts/fft  mask(fft){n_streams=1, FFTSize=9, n_inputs=3, input_bit_width=18, bin_pt_in=0, coeff_bit_width=18, async=off, unscramble=on, add_latency=2, mult_latency=2, bram_latency=2, conv_latency=1, quantization=Round  (unbiased: +/- Inf), overflow=Wrap, delays_bit_limit=8, coeffs_bit_limit=9, coeff_sharing=off, coeff_decimation=off, coeff_generation=on, cal_bits=9, n_bits_rotation=25, max_fanout=4, mult_spec=2, bitgrowth=off, max_bits=19, hardcode_shifts=off, shift_schedule=[], dsp48_adders=on}
      mask prompts: n_streams "Number input streams"; FFTSize "Size of FFT: (2^? pts)"; n_inputs "Number of Simultaneous Inputs: (2^?)"; input_bit_width "Input bit width"; bin_pt_in "Input binary point"; coeff_bit_width "Coefficient Bit Width"; async "Asynchronous operation"; unscramble "Unscramble output (ie, put channels in canonical order)"; add_latency "Add Latency"; mult_latency "Mult Latency"; bram_latency "BRAM Latency"; conv_latency "Convert Latency"; quantization "Quantization Behavior"; overflow "Overflow Behavior"; delays_bit_limit "Number bits above which to store stage's delays in BRAM (2^? bits)"; coeffs_bit_limit "Number bits above which to store stage's coefficients in BRAM (2^? bits)"; coeff_sharing "BRAM sharing in coeff storage"; coeff_decimation "Store a fraction of coeff factors where useful"; coeff_generation "Generate coeffs with multipliers where useful"; cal_bits "Number calibration locations when generating coeffs (2^?)"; n_bits_rotation "Feedback rotation vector resolution"; max_fanout "Maximum fanout"; mult_spec "Multiplier impl. (0=core, 1=embedded, 2=behavioural) (left=1st stage, or just one value)"; bitgrowth "Bitgrowth instead of shifting"; max_bits "Max bits to grow to"; hardcode_shifts "Hardcode shift schedule"; shift_schedule "Shift schedule"; dsp48_adders "DSP48 adders in butterfly"
      mask help: A complex FFT.
      mask init:
      | fft_init(gcb, ...
      |     'n_streams', n_streams, ...
      |     'FFTSize', FFTSize, ...
      |     'n_inputs', n_inputs, ...
      |     'input_bit_width', input_bit_width, ...
      |     'coeff_bit_width', coeff_bit_width, ...
      |     'async', async, ...
      |     'unscramble', unscramble, ...
      |     'add_latency', add_latency, ...
      |     'mult_latency', mult_latency, ...
      |     'bram_latency', bram_latency, ...
      |     'conv_latency', conv_latency, ...
      |     'quantization', quantization, ...
      |     'overflow', overflow, ...
      |     'delays_bit_limit', delays_bit_limit, ...
      |     'coeffs_bit_limit', coeffs_bit_limit, ...
      |     'coeff_sharing', coeff_sharing, ...
      |     'coeff_decimation', coeff_decimation, ...
      |     'coeff_generation', coeff_generation, ...
      |     'cal_bits', cal_bits, ...
      |     'n_bits_rotation', n_bits_rotation, ...
      |     'max_fanout', max_fanout, ...   
      |     'mult_spec', mult_spec, ...
      |     'bitgrowth', bitgrowth, ...
      |     'hardcode_shifts', hardcode_shifts, ...
      |     'shift_schedule', shift_schedule, ...
      |     'dsp48_adders', dsp48_adders);
      settings: AttributesFormatString=|
      | 9 stages
      | (18,18)
      | Round  (unbiased: +/- Inf)
      | Wrap
      mask Help: eval('xlWeb(''http://casper.berkeley.edu/wiki/Fft'')')
      mask TypeOptions quantization: Truncate | Round  (unbiased: +/- Inf) | Round  (unbiased: Even Values)
      mask TypeOptions overflow: Wrap | Saturate | Error
      mask Callback hardcode_shifts:
      | hardcode_shifts = get_param(gcb, 'hardcode_shifts');
      | set_param_state(gcb, 'shift_schedule', hardcode_shifts);
      mask Callback dsp48_adders: fft_callback_dsp48_adders(gcb);
  fft_wideband_real : Subsystem  Tag=casper:fft_wideband_real  AncestorBlock=casper_library_ffts/fft_wideband_real  mask(fft_wideband_real){n_streams=1, FFTSize=8, n_inputs=4, input_bit_width=18, bin_pt_in=17, coeff_bit_width=18, unscramble=on, async=off, floating_point=off, float_type=single, exp_width=8, frac_width=24, add_latency=1, mult_latency=3, bram_latency=3, conv_latency=3, input_latency=1, biplex_direct_latency=1, add_pipe_latency=0, mult_pipe_latency=0, quantization=Round  (unbiased: +/- Inf), overflow=Wrap, delays_bit_limit=8, coeffs_bit_limit=8, coeff_sharing=off, coeff_decimation=off, coeff_generation=off, cal_bits=1, n_bits_rotation=25, mult_spec=2, max_fanout=4, bitgrowth=off, max_bits=19, hardcode_shifts=off, shift_schedule=[], dsp48_adders=off}
      mask prompts: n_streams "Number simultaneous streams"; FFTSize "Size of FFT: (2^? pts)"; n_inputs "Number of Simultaneous Inputs: (2^?)"; input_bit_width "Input Bit Width"; bin_pt_in "Input binary point"; coeff_bit_width "Coefficient Bit Width"; unscramble "Unscramble output (ie, put channels in canonical order)"; async "Asynchronous operation"; floating_point "floating point"; float_type "float type"; exp_width "exponent width"; frac_width "fraction width"; add_latency "Add Latency"; mult_latency "Mult Latency"; bram_latency "BRAM Latency"; conv_latency "Convert Latency"; input_latency "Input Latency"; biplex_direct_latency "Latency between biplexes and fft_direct"; add_pipe_latency "Add Interface Pipeline Latency"; mult_pipe_latency "CMult Pipeline Latency"; quantization "Quantization Behavior"; overflow "Overflow Behavior"; delays_bit_limit "Number bits above which to store stage's delays in BRAM (2^? bits)"; coeffs_bit_limit "Number bits above which to store stage's coefficients in BRAM (2^? bits)"; coeff_sharing "BRAM sharing in coeff storage"; coeff_decimation "Store a fraction of coeff factors where useful"; coeff_generation "Generate coeffs with multipliers where useful"; cal_bits "Number calibration locations when generating coeffs (2^?)"; n_bits_rotation "Feedback rotation vector resolution"; mult_spec "Multiplier impl. (0=core, 1=embedded, 2=behavioural) (left=1st stage, or just one value)"; max_fanout "Maximum fanout"; bitgrowth "Bitgrowth instead of shifting"; max_bits "Max bits to grow to"; hardcode_shifts "Hardcode shift schedule"; shift_schedule "Shift schedule"; dsp48_adders "DSP48 adders in butterfly"
      mask help: A real-sampled wideband FFT.
      mask init:
      | fft_wideband_real_init(gcb, ...
      |     'n_streams', n_streams, ...
      |     'FFTSize', FFTSize, ...
      |     'n_inputs', n_inputs, ...
      |     'input_bit_width', input_bit_width, ...
      |     'bin_pt_in', bin_pt_in, ...
      |     'coeff_bit_width', coeff_bit_width, ...
      |     'floating_point', floating_point, ...
      |     'float_type', float_type, ...
      |     'exp_width', exp_width, ...
      |     'frac_width', frac_width, ...
      |     'unscramble', unscramble, ...
      |     'async', async, ...
      |     'add_latency', add_latency, ...
      |     'mult_latency', mult_latency, ...
      |     'bram_latency', bram_latency, ...
      |     'conv_latency', conv_latency, ...
      |     'input_latency', input_latency, ...
      |     'add_pipe_latency', add_pipe_latency, ...
      |     'mult_pipe_latency', mult_pipe_latency, ...
      |     'biplex_direct_latency', biplex_direct_latency, ...
      |     'quantization', quantization, ...
      |     'overflow', overflow, ...
      |     'delays_bit_limit', delays_bit_limit, ...
      |     'coeffs_bit_limit', coeffs_bit_limit, ...
      |     'coeff_sharing', coeff_sharing, ...
      |     'coeff_decimation', coeff_decimation, ...
      |     'coeff_generation', coeff_generation, ...
      |     'cal_bits', cal_bits, ...
      |     'n_bits_rotation', n_bits_rotation, ...
      |     'max_fanout', max_fanout, ...   
      |     'mult_spec', mult_spec, ...
      |     'bitgrowth', bitgrowth, ...
      |     'max_bits', max_bits, ...
      |     'hardcode_shifts', hardcode_shifts, ...
      |     'shift_schedule', shift_schedule, ...
      |     'dsp48_adders', dsp48_adders);
      settings: AttributesFormatString=|
      | 8 stages
      | (18,18)
      | Round  (unbiased: +/- Inf)
      | Wrap
      mask Help: eval('xlWeb(''http://casper.berkeley.edu/wiki/Fft_wideband_real'')')
      mask Callback floating_point:
      | onoff = get_param(gcb, 'floating_point');
      | if strcmp(onoff,'on')
      |     enable_fixpt = 'off';
      |     set_param_state(gcb, 'float_type', 'on')
      | 
      |     f_type = get_param(gcb, 'float_type')
      |     if strcmp(f_type,'custom')
      |         set_param_state(gcb, 'exp_width', 'on')
      |         set_param_state(gcb, 'frac_width', 'on')
      |     else
      |         set_param_state(gcb, 'exp_width', 'off')
      |         set_param_state(gcb, 'frac_width', 'off')
      |     end
      | 
      | 
      | else
      |     enable_fixpt = 'on';
      |     set_param_state(gcb, 'float_type', 'off')
      |     set_param_state(gcb, 'exp_width', 'off')
      |     set_param_state(gcb, 'frac_width', 'off')
      | end
      | 
      | set_param_state(gcb, 'input_bit_width', enable_fixpt)
      | set_param_state(gcb, 'bin_pt_in', enable_fixpt)
      | set_param_state(gcb, 'coeff_bit_width', enable_fixpt)
      mask TypeOptions float_type: single | custom
      mask Callback float_type:
      | f_type = get_param(gcb, 'float_type');
      | if strcmp(f_type,'custom')
      |     set_param_state(gcb, 'exp_width', 'on')
      |     set_param_state(gcb, 'frac_width', 'on')
      | else
      |     set_param_state(gcb, 'exp_width', 'off')
      |     set_param_state(gcb, 'frac_width', 'off')
      | end
      mask TypeOptions quantization: Truncate | Round  (unbiased: +/- Inf) | Round  (unbiased: Even Values)
      mask TypeOptions overflow: Wrap | Saturate | Error
      mask Callback hardcode_shifts:
      | hardcode_shifts = get_param(gcb, 'hardcode_shifts');
      | set_param_state(gcb, 'shift_schedule', hardcode_shifts);
      mask Callback dsp48_adders: fft_callback_dsp48_adders(gcb);
      mask DialogControl ParameterTabVar0 Prompt: Basic
      mask DialogControl ParameterTabVar01 Prompt: Latency
      mask DialogControl ParameterTabVar012 Prompt: Implementation
  munge1 : Subsystem  AncestorBlock=casper_library_flow_control/munge  mask(munge){divisions=16, div_size=[16 16 16 16 16 16 16 16 16 16 16 16 16 16 16 16], order=[15 14 13 12 11 10 9 8 7 6 5 4 3 2 1 0], arith_type_out=Unsigned, bin_pt_out=0}
      mask prompts: divisions "Number of divisions"; div_size "Division size (bits)"; order "Division packing order"; arith_type_out "Output arithmetic type"; bin_pt_out "Output binary point"
      mask help: Splits an input bus into the specified number of divisions and then recombines them in the order specified (most significant division = 0,least = number divisions-1)
      mask init:
      | munge_init(gcb, ...
      |     'divisions', divisions, ...
      |     'div_size', div_size, ...
      |     'order', order, ...
      |     'arith_type_out', arith_type_out, ...
      |     'bin_pt_out', bin_pt_out);
      settings: AttributesFormatString=|
      | split:[16 16 16 16 16 16 16 16 16 16 16 16 16 16 16 16]
      | join:[15 14 13 12 11 10 9 8 7 6 5 4 3 2 1 0]
      | Unsigned [256,0]
      mask TypeOptions arith_type_out: Unsigned | Signed  (2's comp) | Floating-point
  munge2 : Subsystem  AncestorBlock=casper_library_flow_control/munge  mask(munge){divisions=8, div_size=[36 36 36 36 36 36 36 36], order=[7 6 5 4 3 2 1 0], arith_type_out=Unsigned, bin_pt_out=0}
      mask prompts: divisions "Number of divisions"; div_size "Division size (bits)"; order "Division packing order"; arith_type_out "Output arithmetic type"; bin_pt_out "Output binary point"
      mask help: Splits an input bus into the specified number of divisions and then recombines them in the order specified (most significant division = 0,least = number divisions-1)
      mask init:
      | munge_init(gcb, ...
      |     'divisions', divisions, ...
      |     'div_size', div_size, ...
      |     'order', order, ...
      |     'arith_type_out', arith_type_out, ...
      |     'bin_pt_out', bin_pt_out);
      settings: AttributesFormatString=|
      | split:[36 36 36 36 36 36 36 36]
      | join:[7 6 5 4 3 2 1 0]
      | Unsigned [288,0]
      mask TypeOptions arith_type_out: Unsigned | Signed  (2's comp) | Floating-point
  pfb_fir_real7 : Subsystem  Tag=casper:pfb_fir_real  AncestorBlock=casper_library_pfbs/pfb_fir_real  mask(pfb_fir_real){PFBSize=8, TotalTaps=4, WindowType=hamming, n_inputs=4, n_pol_blocks=1, MakeBiplex=off, BitWidthIn=16, BitWidthOut=18, CoeffBitWidth=16, CoeffDistMem=off, add_latency=1, mult_latency=2, bram_latency=2, fan_latency=1, conv_latency=1, quantization=Round  (unbiased: Even Values), fwidth=2, mult_spec=2, adder_folding=on, adder_imp=Fabric, coeffs_share=off}
      mask prompts: PFBSize "Size of PFB: (2^? pnts)"; TotalTaps "Total Number of Taps:"; WindowType "Windowing Function:"; n_inputs "Number of Simultaneous Inputs: (2^?)"; n_pol_blocks "Number of independent input streams (I.e., number of different polarizations)"; MakeBiplex "Make Biplex?"; BitWidthIn "Input Bitwidth:"; BitWidthOut "Output Bitwidth:"; CoeffBitWidth "Coefficient Bitwidth:"; CoeffDistMem "Use Distributed Memory for Coeffs"; add_latency "Add Latency"; mult_latency "Mult Latency"; bram_latency "BRAM Latency"; fan_latency "Fanout latency"; conv_latency "Convert latency"; quantization "Quantization Behavior"; fwidth "Bin Width Scaling (normal=1)"; mult_spec "Multiplier specification (0=core, 1=embedded, 2=behavioural) (left=1st tap, or just one value)"; adder_folding "Fold adders into DSPs"; adder_imp "Adder implementation"; coeffs_share "Share coefficients between polarisations (use less BRAM)?"
      mask help:
      | Fold adders into DSPs: Causes adders to be absorbed into DSP blocks (supported in Virtex5)
      | Adder implementation: Cores using Fabric or DSP48 or behavioral HDL
      mask init:
      | pfb_fir_real_init(gcb, ...
      |     'PFBSize', PFBSize, ...
      |     'TotalTaps', TotalTaps, ...
      |     'WindowType', WindowType, ...
      |     'n_inputs', n_inputs, ...
      |     'MakeBiplex', MakeBiplex, ...
      |     'BitWidthIn', BitWidthIn, ...
      |     'BitWidthOut', BitWidthOut, ...
      |     'CoeffBitWidth', CoeffBitWidth, ...
      |     'CoeffDistMem', CoeffDistMem, ...
      |     'add_latency', add_latency, ...
      |     'mult_latency', mult_latency, ...
      |     'bram_latency', bram_latency, ...
      |     'fan_latency', fan_latency, ...
      |     'conv_latency', conv_latency, ...
      |     'quantization', quantization, ...
      |     'fwidth', fwidth, ...
      |     'mult_spec', mult_spec, ...
      |     'adder_folding', adder_folding, ...
      |     'adder_imp', adder_imp, ...
      |     'coeffs_share', coeffs_share);
      settings: AttributesFormatString=taps=4, add_latency=1
      mask Help: eval('xlWeb(''http://casper.berkeley.edu/wiki/Pfb_fir_real'')')
      mask Callback TotalTaps:
      | %num_taps = eval(get_param(gcb, 'TotalTaps'));
      | %old_vec = eval(get_param(gcb, 'mult_spec'));=-0l
      | 
      | %vec = 2.*ones(1,num_taps);
      | %old_size = length(old_vec);
      | 
      | %if(old_size <= num_taps),
      | %    new_size = old_size;
      | %else,
      | %    new_size = num_taps;
      | %end
      | 
      | %for n = 1:new_size, vec(n) = old_vec(n); end
      | %set_param(gcb, 'mult_spec', mat2str(vec));
      mask TypeOptions WindowType: bartlett | barthannwin | blackman | blackmanharris | bohamwin | chebwin | flattopwin | gausswin | hamming | hann | kaiser | nuttallwin | parzenwin | rectwin | tukeywin | triang | userwindow
      mask TypeOptions quantization: Truncate | Round  (unbiased: +/- Inf) | Round  (unbiased: Even Values)
      mask TypeOptions adder_imp: Behavioral | Fabric | DSP48
  pipeline : Subsystem  AncestorBlock=casper_library_delays/pipeline  mask(pipeline){csp_latency=2}
      mask prompts: csp_latency "Latency"
      mask help:
      | An explicitly laid-out delay line to avoid mapping to SRL16s
      | for use in pipelining to help achieve timing closure.
      mask init:
      | pipeline_init(gcb,'latency',csp_latency);
      settings: AttributesFormatString=Latency = %<latency>
      mask Display:
      | port_label('input', 1, 'd');
      | port_label('output', 1, 'q');
      | disp(['Z^-', num2str(csp_latency)]);
  pipeline1 : Subsystem  AncestorBlock=casper_library_delays/pipeline  mask(pipeline){csp_latency=2}
      mask prompts: csp_latency "Latency"
      mask help:
      | An explicitly laid-out delay line to avoid mapping to SRL16s
      | for use in pipelining to help achieve timing closure.
      mask init:
      | pipeline_init(gcb,'latency',csp_latency);
      settings: AttributesFormatString=Latency = %<latency>
      mask Display:
      | port_label('input', 1, 'd');
      | port_label('output', 1, 'q');
      | disp(['Z^-', num2str(csp_latency)]);
  pipeline100 : Subsystem  AncestorBlock=casper_library_delays/pipeline  mask(pipeline){csp_latency=1}
      mask prompts: csp_latency "Latency"
      mask help:
      | An explicitly laid-out delay line to avoid mapping to SRL16s
      | for use in pipelining to help achieve timing closure.
      mask init:
      | pipeline_init(gcb,'latency',csp_latency);
      settings: AttributesFormatString=Latency = %<latency>
      mask Display:
      | port_label('input', 1, 'd');
      | port_label('output', 1, 'q');
      | disp(['Z^-', num2str(csp_latency)]);
  pipeline101 : Subsystem  AncestorBlock=casper_library_delays/pipeline  mask(pipeline){csp_latency=1}
      mask prompts: csp_latency "Latency"
      mask help:
      | An explicitly laid-out delay line to avoid mapping to SRL16s
      | for use in pipelining to help achieve timing closure.
      mask init:
      | pipeline_init(gcb,'latency',csp_latency);
      settings: AttributesFormatString=Latency = %<latency>
      mask Display:
      | port_label('input', 1, 'd');
      | port_label('output', 1, 'q');
      | disp(['Z^-', num2str(csp_latency)]);
  pipeline102 : Subsystem  AncestorBlock=casper_library_delays/pipeline  mask(pipeline){csp_latency=1}
      mask prompts: csp_latency "Latency"
      mask help:
      | An explicitly laid-out delay line to avoid mapping to SRL16s
      | for use in pipelining to help achieve timing closure.
      mask init:
      | pipeline_init(gcb,'latency',csp_latency);
      settings: AttributesFormatString=Latency = %<latency>
      mask Display:
      | port_label('input', 1, 'd');
      | port_label('output', 1, 'q');
      | disp(['Z^-', num2str(csp_latency)]);
  pipeline103 : Subsystem  AncestorBlock=casper_library_delays/pipeline  mask(pipeline){csp_latency=1}
      mask prompts: csp_latency "Latency"
      mask help:
      | An explicitly laid-out delay line to avoid mapping to SRL16s
      | for use in pipelining to help achieve timing closure.
      mask init:
      | pipeline_init(gcb,'latency',csp_latency);
      settings: AttributesFormatString=Latency = %<latency>
      mask Display:
      | port_label('input', 1, 'd');
      | port_label('output', 1, 'q');
      | disp(['Z^-', num2str(csp_latency)]);
  pipeline104 : Subsystem  AncestorBlock=casper_library_delays/pipeline  mask(pipeline){csp_latency=1}
      mask prompts: csp_latency "Latency"
      mask help:
      | An explicitly laid-out delay line to avoid mapping to SRL16s
      | for use in pipelining to help achieve timing closure.
      mask init:
      | pipeline_init(gcb,'latency',csp_latency);
      settings: AttributesFormatString=Latency = %<latency>
      mask Display:
      | port_label('input', 1, 'd');
      | port_label('output', 1, 'q');
      | disp(['Z^-', num2str(csp_latency)]);
  pipeline105 : Subsystem  AncestorBlock=casper_library_delays/pipeline  mask(pipeline){csp_latency=1}
      mask prompts: csp_latency "Latency"
      mask help:
      | An explicitly laid-out delay line to avoid mapping to SRL16s
      | for use in pipelining to help achieve timing closure.
      mask init:
      | pipeline_init(gcb,'latency',csp_latency);
      settings: AttributesFormatString=Latency = %<latency>
      mask Display:
      | port_label('input', 1, 'd');
      | port_label('output', 1, 'q');
      | disp(['Z^-', num2str(csp_latency)]);
  pipeline106 : Subsystem  AncestorBlock=casper_library_delays/pipeline  mask(pipeline){csp_latency=1}
      mask prompts: csp_latency "Latency"
      mask help:
      | An explicitly laid-out delay line to avoid mapping to SRL16s
      | for use in pipelining to help achieve timing closure.
      mask init:
      | pipeline_init(gcb,'latency',csp_latency);
      settings: AttributesFormatString=Latency = %<latency>
      mask Display:
      | port_label('input', 1, 'd');
      | port_label('output', 1, 'q');
      | disp(['Z^-', num2str(csp_latency)]);
  pipeline2 : Subsystem  AncestorBlock=casper_library_delays/pipeline  mask(pipeline){csp_latency=2}
      mask prompts: csp_latency "Latency"
      mask help:
      | An explicitly laid-out delay line to avoid mapping to SRL16s
      | for use in pipelining to help achieve timing closure.
      mask init:
      | pipeline_init(gcb,'latency',csp_latency);
      settings: AttributesFormatString=Latency = %<latency>
      mask Display:
      | port_label('input', 1, 'd');
      | port_label('output', 1, 'q');
      | disp(['Z^-', num2str(csp_latency)]);
  pipeline54 : Subsystem  AncestorBlock=casper_library_delays/pipeline  mask(pipeline){csp_latency=1}
      mask prompts: csp_latency "Latency"
      mask help:
      | An explicitly laid-out delay line to avoid mapping to SRL16s
      | for use in pipelining to help achieve timing closure.
      mask init:
      | pipeline_init(gcb,'latency',csp_latency);
      settings: AttributesFormatString=Latency = %<latency>
      mask Display:
      | port_label('input', 1, 'd');
      | port_label('output', 1, 'q');
      | disp(['Z^-', num2str(csp_latency)]);
  pipeline55 : Subsystem  AncestorBlock=casper_library_delays/pipeline  mask(pipeline){csp_latency=1}
      mask prompts: csp_latency "Latency"
      mask help:
      | An explicitly laid-out delay line to avoid mapping to SRL16s
      | for use in pipelining to help achieve timing closure.
      mask init:
      | pipeline_init(gcb,'latency',csp_latency);
      settings: AttributesFormatString=Latency = %<latency>
      mask Display:
      | port_label('input', 1, 'd');
      | port_label('output', 1, 'q');
      | disp(['Z^-', num2str(csp_latency)]);
  pipeline56 : Subsystem  AncestorBlock=casper_library_delays/pipeline  mask(pipeline){csp_latency=1}
      mask prompts: csp_latency "Latency"
      mask help:
      | An explicitly laid-out delay line to avoid mapping to SRL16s
      | for use in pipelining to help achieve timing closure.
      mask init:
      | pipeline_init(gcb,'latency',csp_latency);
      settings: AttributesFormatString=Latency = %<latency>
      mask Display:
      | port_label('input', 1, 'd');
      | port_label('output', 1, 'q');
      | disp(['Z^-', num2str(csp_latency)]);
  pipeline57 : Subsystem  AncestorBlock=casper_library_delays/pipeline  mask(pipeline){csp_latency=1}
      mask prompts: csp_latency "Latency"
      mask help:
      | An explicitly laid-out delay line to avoid mapping to SRL16s
      | for use in pipelining to help achieve timing closure.
      mask init:
      | pipeline_init(gcb,'latency',csp_latency);
      settings: AttributesFormatString=Latency = %<latency>
      mask Display:
      | port_label('input', 1, 'd');
      | port_label('output', 1, 'q');
      | disp(['Z^-', num2str(csp_latency)]);
  pipeline58 : Subsystem  AncestorBlock=casper_library_delays/pipeline  mask(pipeline){csp_latency=1}
      mask prompts: csp_latency "Latency"
      mask help:
      | An explicitly laid-out delay line to avoid mapping to SRL16s
      | for use in pipelining to help achieve timing closure.
      mask init:
      | pipeline_init(gcb,'latency',csp_latency);
      settings: AttributesFormatString=Latency = %<latency>
      mask Display:
      | port_label('input', 1, 'd');
      | port_label('output', 1, 'q');
      | disp(['Z^-', num2str(csp_latency)]);
  pipeline60 : Subsystem  AncestorBlock=casper_library_delays/pipeline  mask(pipeline){csp_latency=1}
      mask prompts: csp_latency "Latency"
      mask help:
      | An explicitly laid-out delay line to avoid mapping to SRL16s
      | for use in pipelining to help achieve timing closure.
      mask init:
      | pipeline_init(gcb,'latency',csp_latency);
      settings: AttributesFormatString=Latency = %<latency>
      mask Display:
      | port_label('input', 1, 'd');
      | port_label('output', 1, 'q');
      | disp(['Z^-', num2str(csp_latency)]);
  pipeline61 : Subsystem  AncestorBlock=casper_library_delays/pipeline  mask(pipeline){csp_latency=1}
      mask prompts: csp_latency "Latency"
      mask help:
      | An explicitly laid-out delay line to avoid mapping to SRL16s
      | for use in pipelining to help achieve timing closure.
      mask init:
      | pipeline_init(gcb,'latency',csp_latency);
      settings: AttributesFormatString=Latency = %<latency>
      mask Display:
      | port_label('input', 1, 'd');
      | port_label('output', 1, 'q');
      | disp(['Z^-', num2str(csp_latency)]);
  pipeline62 : Subsystem  AncestorBlock=casper_library_delays/pipeline  mask(pipeline){csp_latency=1}
      mask prompts: csp_latency "Latency"
      mask help:
      | An explicitly laid-out delay line to avoid mapping to SRL16s
      | for use in pipelining to help achieve timing closure.
      mask init:
      | pipeline_init(gcb,'latency',csp_latency);
      settings: AttributesFormatString=Latency = %<latency>
      mask Display:
      | port_label('input', 1, 'd');
      | port_label('output', 1, 'q');
      | disp(['Z^-', num2str(csp_latency)]);
  pipeline63 : Subsystem  AncestorBlock=casper_library_delays/pipeline  mask(pipeline){csp_latency=1}
      mask prompts: csp_latency "Latency"
      mask help:
      | An explicitly laid-out delay line to avoid mapping to SRL16s
      | for use in pipelining to help achieve timing closure.
      mask init:
      | pipeline_init(gcb,'latency',csp_latency);
      settings: AttributesFormatString=Latency = %<latency>
      mask Display:
      | port_label('input', 1, 'd');
      | port_label('output', 1, 'q');
      | disp(['Z^-', num2str(csp_latency)]);
  pipeline64 : Subsystem  AncestorBlock=casper_library_delays/pipeline  mask(pipeline){csp_latency=1}
      mask prompts: csp_latency "Latency"
      mask help:
      | An explicitly laid-out delay line to avoid mapping to SRL16s
      | for use in pipelining to help achieve timing closure.
      mask init:
      | pipeline_init(gcb,'latency',csp_latency);
      settings: AttributesFormatString=Latency = %<latency>
      mask Display:
      | port_label('input', 1, 'd');
      | port_label('output', 1, 'q');
      | disp(['Z^-', num2str(csp_latency)]);
  pipeline65 : Subsystem  AncestorBlock=casper_library_delays/pipeline  mask(pipeline){csp_latency=1}
      mask prompts: csp_latency "Latency"
      mask help:
      | An explicitly laid-out delay line to avoid mapping to SRL16s
      | for use in pipelining to help achieve timing closure.
      mask init:
      | pipeline_init(gcb,'latency',csp_latency);
      settings: AttributesFormatString=Latency = %<latency>
      mask Display:
      | port_label('input', 1, 'd');
      | port_label('output', 1, 'q');
      | disp(['Z^-', num2str(csp_latency)]);
  pipeline66 : Subsystem  AncestorBlock=casper_library_delays/pipeline  mask(pipeline){csp_latency=1}
      mask prompts: csp_latency "Latency"
      mask help:
      | An explicitly laid-out delay line to avoid mapping to SRL16s
      | for use in pipelining to help achieve timing closure.
      mask init:
      | pipeline_init(gcb,'latency',csp_latency);
      settings: AttributesFormatString=Latency = %<latency>
      mask Display:
      | port_label('input', 1, 'd');
      | port_label('output', 1, 'q');
      | disp(['Z^-', num2str(csp_latency)]);
  pipeline67 : Subsystem  AncestorBlock=casper_library_delays/pipeline  mask(pipeline){csp_latency=1}
      mask prompts: csp_latency "Latency"
      mask help:
      | An explicitly laid-out delay line to avoid mapping to SRL16s
      | for use in pipelining to help achieve timing closure.
      mask init:
      | pipeline_init(gcb,'latency',csp_latency);
      settings: AttributesFormatString=Latency = %<latency>
      mask Display:
      | port_label('input', 1, 'd');
      | port_label('output', 1, 'q');
      | disp(['Z^-', num2str(csp_latency)]);
  pipeline68 : Subsystem  AncestorBlock=casper_library_delays/pipeline  mask(pipeline){csp_latency=1}
      mask prompts: csp_latency "Latency"
      mask help:
      | An explicitly laid-out delay line to avoid mapping to SRL16s
      | for use in pipelining to help achieve timing closure.
      mask init:
      | pipeline_init(gcb,'latency',csp_latency);
      settings: AttributesFormatString=Latency = %<latency>
      mask Display:
      | port_label('input', 1, 'd');
      | port_label('output', 1, 'q');
      | disp(['Z^-', num2str(csp_latency)]);
  pipeline69 : Subsystem  AncestorBlock=casper_library_delays/pipeline  mask(pipeline){csp_latency=1}
      mask prompts: csp_latency "Latency"
      mask help:
      | An explicitly laid-out delay line to avoid mapping to SRL16s
      | for use in pipelining to help achieve timing closure.
      mask init:
      | pipeline_init(gcb,'latency',csp_latency);
      settings: AttributesFormatString=Latency = %<latency>
      mask Display:
      | port_label('input', 1, 'd');
      | port_label('output', 1, 'q');
      | disp(['Z^-', num2str(csp_latency)]);
  pipeline71 : Subsystem  AncestorBlock=casper_library_delays/pipeline  mask(pipeline){csp_latency=1}
      mask prompts: csp_latency "Latency"
      mask help:
      | An explicitly laid-out delay line to avoid mapping to SRL16s
      | for use in pipelining to help achieve timing closure.
      mask init:
      | pipeline_init(gcb,'latency',csp_latency);
      settings: AttributesFormatString=Latency = %<latency>
      mask Display:
      | port_label('input', 1, 'd');
      | port_label('output', 1, 'q');
      | disp(['Z^-', num2str(csp_latency)]);
  pipeline72 : Subsystem  AncestorBlock=casper_library_delays/pipeline  mask(pipeline){csp_latency=1}
      mask prompts: csp_latency "Latency"
      mask help:
      | An explicitly laid-out delay line to avoid mapping to SRL16s
      | for use in pipelining to help achieve timing closure.
      mask init:
      | pipeline_init(gcb,'latency',csp_latency);
      settings: AttributesFormatString=Latency = %<latency>
      mask Display:
      | port_label('input', 1, 'd');
      | port_label('output', 1, 'q');
      | disp(['Z^-', num2str(csp_latency)]);
  pipeline73 : Subsystem  AncestorBlock=casper_library_delays/pipeline  mask(pipeline){csp_latency=1}
      mask prompts: csp_latency "Latency"
      mask help:
      | An explicitly laid-out delay line to avoid mapping to SRL16s
      | for use in pipelining to help achieve timing closure.
      mask init:
      | pipeline_init(gcb,'latency',csp_latency);
      settings: AttributesFormatString=Latency = %<latency>
      mask Display:
      | port_label('input', 1, 'd');
      | port_label('output', 1, 'q');
      | disp(['Z^-', num2str(csp_latency)]);
  pipeline74 : Subsystem  AncestorBlock=casper_library_delays/pipeline  mask(pipeline){csp_latency=1}
      mask prompts: csp_latency "Latency"
      mask help:
      | An explicitly laid-out delay line to avoid mapping to SRL16s
      | for use in pipelining to help achieve timing closure.
      mask init:
      | pipeline_init(gcb,'latency',csp_latency);
      settings: AttributesFormatString=Latency = %<latency>
      mask Display:
      | port_label('input', 1, 'd');
      | port_label('output', 1, 'q');
      | disp(['Z^-', num2str(csp_latency)]);
  pipeline75 : Subsystem  AncestorBlock=casper_library_delays/pipeline  mask(pipeline){csp_latency=1}
      mask prompts: csp_latency "Latency"
      mask help:
      | An explicitly laid-out delay line to avoid mapping to SRL16s
      | for use in pipelining to help achieve timing closure.
      mask init:
      | pipeline_init(gcb,'latency',csp_latency);
      settings: AttributesFormatString=Latency = %<latency>
      mask Display:
      | port_label('input', 1, 'd');
      | port_label('output', 1, 'q');
      | disp(['Z^-', num2str(csp_latency)]);
  pipeline76 : Subsystem  AncestorBlock=casper_library_delays/pipeline  mask(pipeline){csp_latency=1}
      mask prompts: csp_latency "Latency"
      mask help:
      | An explicitly laid-out delay line to avoid mapping to SRL16s
      | for use in pipelining to help achieve timing closure.
      mask init:
      | pipeline_init(gcb,'latency',csp_latency);
      settings: AttributesFormatString=Latency = %<latency>
      mask Display:
      | port_label('input', 1, 'd');
      | port_label('output', 1, 'q');
      | disp(['Z^-', num2str(csp_latency)]);
  pipeline79 : Subsystem  AncestorBlock=casper_library_delays/pipeline  mask(pipeline){csp_latency=1}
      mask prompts: csp_latency "Latency"
      mask help:
      | An explicitly laid-out delay line to avoid mapping to SRL16s
      | for use in pipelining to help achieve timing closure.
      mask init:
      | pipeline_init(gcb,'latency',csp_latency);
      settings: AttributesFormatString=Latency = %<latency>
      mask Display:
      | port_label('input', 1, 'd');
      | port_label('output', 1, 'q');
      | disp(['Z^-', num2str(csp_latency)]);
  pipeline80 : Subsystem  AncestorBlock=casper_library_delays/pipeline  mask(pipeline){csp_latency=1}
      mask prompts: csp_latency "Latency"
      mask help:
      | An explicitly laid-out delay line to avoid mapping to SRL16s
      | for use in pipelining to help achieve timing closure.
      mask init:
      | pipeline_init(gcb,'latency',csp_latency);
      settings: AttributesFormatString=Latency = %<latency>
      mask Display:
      | port_label('input', 1, 'd');
      | port_label('output', 1, 'q');
      | disp(['Z^-', num2str(csp_latency)]);
  pipeline81 : Subsystem  AncestorBlock=casper_library_delays/pipeline  mask(pipeline){csp_latency=1}
      mask prompts: csp_latency "Latency"
      mask help:
      | An explicitly laid-out delay line to avoid mapping to SRL16s
      | for use in pipelining to help achieve timing closure.
      mask init:
      | pipeline_init(gcb,'latency',csp_latency);
      settings: AttributesFormatString=Latency = %<latency>
      mask Display:
      | port_label('input', 1, 'd');
      | port_label('output', 1, 'q');
      | disp(['Z^-', num2str(csp_latency)]);
  pipeline82 : Subsystem  AncestorBlock=casper_library_delays/pipeline  mask(pipeline){csp_latency=1}
      mask prompts: csp_latency "Latency"
      mask help:
      | An explicitly laid-out delay line to avoid mapping to SRL16s
      | for use in pipelining to help achieve timing closure.
      mask init:
      | pipeline_init(gcb,'latency',csp_latency);
      settings: AttributesFormatString=Latency = %<latency>
      mask Display:
      | port_label('input', 1, 'd');
      | port_label('output', 1, 'q');
      | disp(['Z^-', num2str(csp_latency)]);
  pipeline83 : Subsystem  AncestorBlock=casper_library_delays/pipeline  mask(pipeline){csp_latency=1}
      mask prompts: csp_latency "Latency"
      mask help:
      | An explicitly laid-out delay line to avoid mapping to SRL16s
      | for use in pipelining to help achieve timing closure.
      mask init:
      | pipeline_init(gcb,'latency',csp_latency);
      settings: AttributesFormatString=Latency = %<latency>
      mask Display:
      | port_label('input', 1, 'd');
      | port_label('output', 1, 'q');
      | disp(['Z^-', num2str(csp_latency)]);
  pipeline84 : Subsystem  AncestorBlock=casper_library_delays/pipeline  mask(pipeline){csp_latency=1}
      mask prompts: csp_latency "Latency"
      mask help:
      | An explicitly laid-out delay line to avoid mapping to SRL16s
      | for use in pipelining to help achieve timing closure.
      mask init:
      | pipeline_init(gcb,'latency',csp_latency);
      settings: AttributesFormatString=Latency = %<latency>
      mask Display:
      | port_label('input', 1, 'd');
      | port_label('output', 1, 'q');
      | disp(['Z^-', num2str(csp_latency)]);
  pipeline85 : Subsystem  AncestorBlock=casper_library_delays/pipeline  mask(pipeline){csp_latency=1}
      mask prompts: csp_latency "Latency"
      mask help:
      | An explicitly laid-out delay line to avoid mapping to SRL16s
      | for use in pipelining to help achieve timing closure.
      mask init:
      | pipeline_init(gcb,'latency',csp_latency);
      settings: AttributesFormatString=Latency = %<latency>
      mask Display:
      | port_label('input', 1, 'd');
      | port_label('output', 1, 'q');
      | disp(['Z^-', num2str(csp_latency)]);
  pipeline86 : Subsystem  AncestorBlock=casper_library_delays/pipeline  mask(pipeline){csp_latency=1}
      mask prompts: csp_latency "Latency"
      mask help:
      | An explicitly laid-out delay line to avoid mapping to SRL16s
      | for use in pipelining to help achieve timing closure.
      mask init:
      | pipeline_init(gcb,'latency',csp_latency);
      settings: AttributesFormatString=Latency = %<latency>
      mask Display:
      | port_label('input', 1, 'd');
      | port_label('output', 1, 'q');
      | disp(['Z^-', num2str(csp_latency)]);
  pipeline87 : Subsystem  AncestorBlock=casper_library_delays/pipeline  mask(pipeline){csp_latency=1}
      mask prompts: csp_latency "Latency"
      mask help:
      | An explicitly laid-out delay line to avoid mapping to SRL16s
      | for use in pipelining to help achieve timing closure.
      mask init:
      | pipeline_init(gcb,'latency',csp_latency);
      settings: AttributesFormatString=Latency = %<latency>
      mask Display:
      | port_label('input', 1, 'd');
      | port_label('output', 1, 'q');
      | disp(['Z^-', num2str(csp_latency)]);
  pipeline88 : Subsystem  AncestorBlock=casper_library_delays/pipeline  mask(pipeline){csp_latency=1}
      mask prompts: csp_latency "Latency"
      mask help:
      | An explicitly laid-out delay line to avoid mapping to SRL16s
      | for use in pipelining to help achieve timing closure.
      mask init:
      | pipeline_init(gcb,'latency',csp_latency);
      settings: AttributesFormatString=Latency = %<latency>
      mask Display:
      | port_label('input', 1, 'd');
      | port_label('output', 1, 'q');
      | disp(['Z^-', num2str(csp_latency)]);
  pipeline89 : Subsystem  AncestorBlock=casper_library_delays/pipeline  mask(pipeline){csp_latency=1}
      mask prompts: csp_latency "Latency"
      mask help:
      | An explicitly laid-out delay line to avoid mapping to SRL16s
      | for use in pipelining to help achieve timing closure.
      mask init:
      | pipeline_init(gcb,'latency',csp_latency);
      settings: AttributesFormatString=Latency = %<latency>
      mask Display:
      | port_label('input', 1, 'd');
      | port_label('output', 1, 'q');
      | disp(['Z^-', num2str(csp_latency)]);
  pipeline90 : Subsystem  AncestorBlock=casper_library_delays/pipeline  mask(pipeline){csp_latency=1}
      mask prompts: csp_latency "Latency"
      mask help:
      | An explicitly laid-out delay line to avoid mapping to SRL16s
      | for use in pipelining to help achieve timing closure.
      mask init:
      | pipeline_init(gcb,'latency',csp_latency);
      settings: AttributesFormatString=Latency = %<latency>
      mask Display:
      | port_label('input', 1, 'd');
      | port_label('output', 1, 'q');
      | disp(['Z^-', num2str(csp_latency)]);
  pipeline91 : Subsystem  AncestorBlock=casper_library_delays/pipeline  mask(pipeline){csp_latency=1}
      mask prompts: csp_latency "Latency"
      mask help:
      | An explicitly laid-out delay line to avoid mapping to SRL16s
      | for use in pipelining to help achieve timing closure.
      mask init:
      | pipeline_init(gcb,'latency',csp_latency);
      settings: AttributesFormatString=Latency = %<latency>
      mask Display:
      | port_label('input', 1, 'd');
      | port_label('output', 1, 'q');
      | disp(['Z^-', num2str(csp_latency)]);
  pipeline92 : Subsystem  AncestorBlock=casper_library_delays/pipeline  mask(pipeline){csp_latency=1}
      mask prompts: csp_latency "Latency"
      mask help:
      | An explicitly laid-out delay line to avoid mapping to SRL16s
      | for use in pipelining to help achieve timing closure.
      mask init:
      | pipeline_init(gcb,'latency',csp_latency);
      settings: AttributesFormatString=Latency = %<latency>
      mask Display:
      | port_label('input', 1, 'd');
      | port_label('output', 1, 'q');
      | disp(['Z^-', num2str(csp_latency)]);
  pipeline93 : Subsystem  AncestorBlock=casper_library_delays/pipeline  mask(pipeline){csp_latency=1}
      mask prompts: csp_latency "Latency"
      mask help:
      | An explicitly laid-out delay line to avoid mapping to SRL16s
      | for use in pipelining to help achieve timing closure.
      mask init:
      | pipeline_init(gcb,'latency',csp_latency);
      settings: AttributesFormatString=Latency = %<latency>
      mask Display:
      | port_label('input', 1, 'd');
      | port_label('output', 1, 'q');
      | disp(['Z^-', num2str(csp_latency)]);
  pipeline94 : Subsystem  AncestorBlock=casper_library_delays/pipeline  mask(pipeline){csp_latency=1}
      mask prompts: csp_latency "Latency"
      mask help:
      | An explicitly laid-out delay line to avoid mapping to SRL16s
      | for use in pipelining to help achieve timing closure.
      mask init:
      | pipeline_init(gcb,'latency',csp_latency);
      settings: AttributesFormatString=Latency = %<latency>
      mask Display:
      | port_label('input', 1, 'd');
      | port_label('output', 1, 'q');
      | disp(['Z^-', num2str(csp_latency)]);
  pipeline95 : Subsystem  AncestorBlock=casper_library_delays/pipeline  mask(pipeline){csp_latency=1}
      mask prompts: csp_latency "Latency"
      mask help:
      | An explicitly laid-out delay line to avoid mapping to SRL16s
      | for use in pipelining to help achieve timing closure.
      mask init:
      | pipeline_init(gcb,'latency',csp_latency);
      settings: AttributesFormatString=Latency = %<latency>
      mask Display:
      | port_label('input', 1, 'd');
      | port_label('output', 1, 'q');
      | disp(['Z^-', num2str(csp_latency)]);
  pipeline96 : Subsystem  AncestorBlock=casper_library_delays/pipeline  mask(pipeline){csp_latency=1}
      mask prompts: csp_latency "Latency"
      mask help:
      | An explicitly laid-out delay line to avoid mapping to SRL16s
      | for use in pipelining to help achieve timing closure.
      mask init:
      | pipeline_init(gcb,'latency',csp_latency);
      settings: AttributesFormatString=Latency = %<latency>
      mask Display:
      | port_label('input', 1, 'd');
      | port_label('output', 1, 'q');
      | disp(['Z^-', num2str(csp_latency)]);
  pipeline97 : Subsystem  AncestorBlock=casper_library_delays/pipeline  mask(pipeline){csp_latency=1}
      mask prompts: csp_latency "Latency"
      mask help:
      | An explicitly laid-out delay line to avoid mapping to SRL16s
      | for use in pipelining to help achieve timing closure.
      mask init:
      | pipeline_init(gcb,'latency',csp_latency);
      settings: AttributesFormatString=Latency = %<latency>
      mask Display:
      | port_label('input', 1, 'd');
      | port_label('output', 1, 'q');
      | disp(['Z^-', num2str(csp_latency)]);
  pipeline98 : Subsystem  AncestorBlock=casper_library_delays/pipeline  mask(pipeline){csp_latency=1}
      mask prompts: csp_latency "Latency"
      mask help:
      | An explicitly laid-out delay line to avoid mapping to SRL16s
      | for use in pipelining to help achieve timing closure.
      mask init:
      | pipeline_init(gcb,'latency',csp_latency);
      settings: AttributesFormatString=Latency = %<latency>
      mask Display:
      | port_label('input', 1, 'd');
      | port_label('output', 1, 'q');
      | disp(['Z^-', num2str(csp_latency)]);
  pipeline99 : Subsystem  AncestorBlock=casper_library_delays/pipeline  mask(pipeline){csp_latency=1}
      mask prompts: csp_latency "Latency"
      mask help:
      | An explicitly laid-out delay line to avoid mapping to SRL16s
      | for use in pipelining to help achieve timing closure.
      mask init:
      | pipeline_init(gcb,'latency',csp_latency);
      settings: AttributesFormatString=Latency = %<latency>
      mask Display:
      | port_label('input', 1, 'd');
      | port_label('output', 1, 'q');
      | disp(['Z^-', num2str(csp_latency)]);
  power{9..16} (8 alike) : casper_library_misc/power  BitWidth=18  add_latency=2  mult_latency=3
      settings: SourceProductName=CASPER DSP Blockset
  q1 : Subsystem  Tag=xps:bram  AncestorBlock=xps_library/Memory/shared_bram  mask{arith_type=Unsigned, addr_width=13, data_width=64, reg_prim_output=on, reg_core_output=on, optimization=Minimum_Area, data_bin_pt=0, init_vals=[0:2^13-1], sample_rate=1}
      mask prompts: arith_type "Output Data Type"; addr_width "Address width"; data_width "Data Width"; reg_prim_output "Register Primitive Output"; reg_core_output "Register Core Output"; data_bin_pt "Data Binary Point"; init_vals "Initial values (simulation only)"; sample_rate "Sample rate"
      mask init:
      | shared_bram_mask;
      mask TypeOptions arith_type: Unsigned | Signed  (2's comp)
      mask TypeOptions data_width: 8 | 16 | 32 | 64 | 128
      mask TypeOptions optimization: Minimum_Area | Low_Power
  q2 : Subsystem  Tag=xps:bram  AncestorBlock=xps_library/Memory/shared_bram  mask{arith_type=Unsigned, addr_width=13, data_width=64, reg_prim_output=on, reg_core_output=on, optimization=Minimum_Area, data_bin_pt=0, init_vals=[0:2^13-1], sample_rate=1}
      mask prompts: arith_type "Output Data Type"; addr_width "Address width"; data_width "Data Width"; reg_prim_output "Register Primitive Output"; reg_core_output "Register Core Output"; data_bin_pt "Data Binary Point"; init_vals "Initial values (simulation only)"; sample_rate "Sample rate"
      mask init:
      | shared_bram_mask;
      mask TypeOptions arith_type: Unsigned | Signed  (2's comp)
      mask TypeOptions data_width: 8 | 16 | 32 | 64 | 128
      mask TypeOptions optimization: Minimum_Area | Low_Power
  q3 : Subsystem  Tag=xps:bram  AncestorBlock=xps_library/Memory/shared_bram  mask{arith_type=Unsigned, addr_width=13, data_width=64, reg_prim_output=on, reg_core_output=on, optimization=Minimum_Area, data_bin_pt=0, init_vals=[0:2^13-1], sample_rate=1}
      mask prompts: arith_type "Output Data Type"; addr_width "Address width"; data_width "Data Width"; reg_prim_output "Register Primitive Output"; reg_core_output "Register Core Output"; data_bin_pt "Data Binary Point"; init_vals "Initial values (simulation only)"; sample_rate "Sample rate"
      mask init:
      | shared_bram_mask;
      mask TypeOptions arith_type: Unsigned | Signed  (2's comp)
      mask TypeOptions data_width: 8 | 16 | 32 | 64 | 128
      mask TypeOptions optimization: Minimum_Area | Low_Power
  q4 : Subsystem  Tag=xps:bram  AncestorBlock=xps_library/Memory/shared_bram  mask{arith_type=Unsigned, addr_width=13, data_width=64, reg_prim_output=on, reg_core_output=on, optimization=Minimum_Area, data_bin_pt=0, init_vals=[0:2^13-1], sample_rate=1}
      mask prompts: arith_type "Output Data Type"; addr_width "Address width"; data_width "Data Width"; reg_prim_output "Register Primitive Output"; reg_core_output "Register Core Output"; data_bin_pt "Data Binary Point"; init_vals "Initial values (simulation only)"; sample_rate "Sample rate"
      mask init:
      | shared_bram_mask;
      mask TypeOptions arith_type: Unsigned | Signed  (2's comp)
      mask TypeOptions data_width: 8 | 16 | 32 | 64 | 128
      mask TypeOptions optimization: Minimum_Area | Low_Power
  q5 : Subsystem  Tag=xps:bram  AncestorBlock=xps_library/Memory/shared_bram  mask{arith_type=Unsigned, addr_width=13, data_width=64, reg_prim_output=on, reg_core_output=on, optimization=Minimum_Area, data_bin_pt=0, init_vals=[0:2^13-1], sample_rate=1}
      mask prompts: arith_type "Output Data Type"; addr_width "Address width"; data_width "Data Width"; reg_prim_output "Register Primitive Output"; reg_core_output "Register Core Output"; data_bin_pt "Data Binary Point"; init_vals "Initial values (simulation only)"; sample_rate "Sample rate"
      mask init:
      | shared_bram_mask;
      mask TypeOptions arith_type: Unsigned | Signed  (2's comp)
      mask TypeOptions data_width: 8 | 16 | 32 | 64 | 128
      mask TypeOptions optimization: Minimum_Area | Low_Power
  q6 : Subsystem  Tag=xps:bram  AncestorBlock=xps_library/Memory/shared_bram  mask{arith_type=Unsigned, addr_width=13, data_width=64, reg_prim_output=on, reg_core_output=on, optimization=Minimum_Area, data_bin_pt=0, init_vals=[0:2^13-1], sample_rate=1}
      mask prompts: arith_type "Output Data Type"; addr_width "Address width"; data_width "Data Width"; reg_prim_output "Register Primitive Output"; reg_core_output "Register Core Output"; data_bin_pt "Data Binary Point"; init_vals "Initial values (simulation only)"; sample_rate "Sample rate"
      mask init:
      | shared_bram_mask;
      mask TypeOptions arith_type: Unsigned | Signed  (2's comp)
      mask TypeOptions data_width: 8 | 16 | 32 | 64 | 128
      mask TypeOptions optimization: Minimum_Area | Low_Power
  q7 : Subsystem  Tag=xps:bram  AncestorBlock=xps_library/Memory/shared_bram  mask{arith_type=Unsigned, addr_width=13, data_width=64, reg_prim_output=on, reg_core_output=on, optimization=Minimum_Area, data_bin_pt=0, init_vals=[0:2^13-1], sample_rate=1}
      mask prompts: arith_type "Output Data Type"; addr_width "Address width"; data_width "Data Width"; reg_prim_output "Register Primitive Output"; reg_core_output "Register Core Output"; data_bin_pt "Data Binary Point"; init_vals "Initial values (simulation only)"; sample_rate "Sample rate"
      mask init:
      | shared_bram_mask;
      mask TypeOptions arith_type: Unsigned | Signed  (2's comp)
      mask TypeOptions data_width: 8 | 16 | 32 | 64 | 128
      mask TypeOptions optimization: Minimum_Area | Low_Power
  q8 : Subsystem  Tag=xps:bram  AncestorBlock=xps_library/Memory/shared_bram  mask{arith_type=Unsigned, addr_width=13, data_width=64, reg_prim_output=on, reg_core_output=on, optimization=Minimum_Area, data_bin_pt=0, init_vals=[0:2^13-1], sample_rate=1}
      mask prompts: arith_type "Output Data Type"; addr_width "Address width"; data_width "Data Width"; reg_prim_output "Register Primitive Output"; reg_core_output "Register Core Output"; data_bin_pt "Data Binary Point"; init_vals "Initial values (simulation only)"; sample_rate "Sample rate"
      mask init:
      | shared_bram_mask;
      mask TypeOptions arith_type: Unsigned | Signed  (2's comp)
      mask TypeOptions data_width: 8 | 16 | 32 | 64 | 128
      mask TypeOptions optimization: Minimum_Area | Low_Power
  rfdc : Subsystem  Tag=xps:rfdc  AncestorBlock=xps_library/ADCs/rfdc  mask(Xilinx RF Data Converter){forceredraw=0, maskopening=1, runinit=0, Tile224_enable=on, t224_enable_mts=off, t224_sample_rate=1600, t224_clk_out=100, t224_enable_pll=on, t224_ref_clk=400, t224_axi_stream_clk=200, t224_QT_adc0_enable=on, t224_QT_adc0_digital_output=Real, t224_QT_adc0_dec_mode=1x, t224_QT_adc0_sample_per_cycle=8, t224_QT_adc0_req_axis_clk=250, t224_QT_adc0_mixer_type=Bypassed, t224_QT_adc0_mixer_mode=Real -> Real, t224_QT_adc0_nco_freq=0, t224_QT_adc0_nco_phase=0, t224_QT_adc0_coarse_freq=0, t224_QT_adc0_nyquist_zone=Zone 1, t224_QT_adc0_cal_mode=Mode 2, t224_QT_adc1_enable=off, t224_QT_adc1_digital_output=Real, t224_QT_adc1_dec_mode=1x, t224_QT_adc1_sample_per_cycle=8, t224_QT_adc1_req_axis_clk=250, t224_QT_adc1_mixer_type=Bypassed, t224_QT_adc1_mixer_mode=Real -> Real, t224_QT_adc1_nco_freq=0, t224_QT_adc1_nco_phase=0, t224_QT_adc1_coarse_freq=0, t224_QT_adc1_nyquist_zone=Zone 1, t224_QT_adc1_cal_mode=Mode 2, t224_QT_adc2_enable=off, t224_QT_adc2_digital_output=Real, t224_QT_adc2_dec_mode=1x, t224_QT_adc2_sample_per_cycle=8, t224_QT_adc2_req_axis_clk=250, t224_QT_adc2_mixer_type=Bypassed, t224_QT_adc2_mixer_mode=Real -> Real, t224_QT_adc2_nco_freq=0, t224_QT_adc2_nco_phase=0, t224_QT_adc2_coarse_freq=0, t224_QT_adc2_nyquist_zone=Zone 1, t224_QT_adc2_cal_mode=Mode 2, t224_QT_adc3_enable=off, t224_QT_adc3_digital_output=Real, t224_QT_adc3_dec_mode=1x, t224_QT_adc3_sample_per_cycle=8, t224_QT_adc3_req_axis_clk=250, t224_QT_adc3_mixer_type=Bypassed, t224_QT_adc3_mixer_mode=Real -> Real, t224_QT_adc3_nco_freq=0, t224_QT_adc3_nco_phase=0, t224_QT_adc3_coarse_freq=0, t224_QT_adc3_nyquist_zone=Zone 1, t224_QT_adc3_cal_mode=Mode 2, t224_DT_adc0_enable=on, t224_DT_adc0_digital_output=Real, t224_DT_adc0_dec_mode=1x, t224_DT_adc0_sample_per_cycle=8, t224_DT_adc0_req_axis_clk=200, t224_DT_adc0_mixer_type=Bypassed, t224_DT_adc0_mixer_mode=Real -> Real, t224_DT_adc0_nco_freq=0, t224_DT_adc0_nco_phase=0, t224_DT_adc0_coarse_freq=0, t224_DT_adc0_nyquist_zone=Zone 1, t224_DT_adc0_cal_mode=Mode 2, t224_DT_adc1_enable=on, t224_DT_adc1_digital_output=Real, t224_DT_adc1_dec_mode=1x, t224_DT_adc1_sample_per_cycle=8, t224_DT_adc1_req_axis_clk=200, t224_DT_adc1_mixer_type=Bypassed, t224_DT_adc1_mixer_mode=Real -> Real, t224_DT_adc1_nco_freq=0, t224_DT_adc1_nco_phase=0, t224_DT_adc1_coarse_freq=0, t224_DT_adc1_nyquist_zone=Zone 1, t224_DT_adc1_cal_mode=Mode 2, Tile225_enable=on, t225_enable_mts=off, t225_sample_rate=1600, t225_clk_out=100, t225_enable_pll=on, t225_ref_clk=400, t225_axi_stream_clk=200, t225_QT_adc0_enable=on, t225_QT_adc0_digital_output=Real, t225_QT_adc0_dec_mode=1x, t225_QT_adc0_sample_per_cycle=8, t225_QT_adc0_req_axis_clk=250, t225_QT_adc0_mixer_type=Bypassed, t225_QT_adc0_mixer_mode=Real -> Real, t225_QT_adc0_nco_freq=0, t225_QT_adc0_nco_phase=0, t225_QT_adc0_coarse_freq=0, t225_QT_adc0_nyquist_zone=Zone 1, t225_QT_adc0_cal_mode=Mode 2, t225_QT_adc1_enable=off, t225_QT_adc1_digital_output=Real, t225_QT_adc1_dec_mode=1x, t225_QT_adc1_sample_per_cycle=8, t225_QT_adc1_req_axis_clk=250, t225_QT_adc1_mixer_type=Bypassed, t225_QT_adc1_mixer_mode=Real -> Real, t225_QT_adc1_nco_freq=0, t225_QT_adc1_nco_phase=0, t225_QT_adc1_coarse_freq=0, t225_QT_adc1_nyquist_zone=Zone 1, t225_QT_adc1_cal_mode=Mode 2, t225_QT_adc2_enable=off, t225_QT_adc2_digital_output=Real, t225_QT_adc2_dec_mode=1x, t225_QT_adc2_sample_per_cycle=8, t225_QT_adc2_req_axis_clk=250, t225_QT_adc2_mixer_type=Bypassed, t225_QT_adc2_mixer_mode=Real -> Real, t225_QT_adc2_nco_freq=0, t225_QT_adc2_nco_phase=0, t225_QT_adc2_coarse_freq=0, t225_QT_adc2_nyquist_zone=Zone 1, t225_QT_adc2_cal_mode=Mode 2, t225_QT_adc3_enable=off, t225_QT_adc3_digital_output=Real, t225_QT_adc3_dec_mode=1x, t225_QT_adc3_sample_per_cycle=8, t225_QT_adc3_req_axis_clk=250, t225_QT_adc3_mixer_type=Bypassed, t225_QT_adc3_mixer_mode=Real -> Real, t225_QT_adc3_nco_freq=0, t225_QT_adc3_nco_phase=0, t225_QT_adc3_coarse_freq=0, t225_QT_adc3_nyquist_zone=Zone 1, t225_QT_adc3_cal_mode=Mode 2, t225_DT_adc0_enable=on, t225_DT_adc0_digital_output=Real, t225_DT_adc0_dec_mode=1x, t225_DT_adc0_sample_per_cycle=8, t225_DT_adc0_req_axis_clk=200, t225_DT_adc0_mixer_type=Bypassed, t225_DT_adc0_mixer_mode=Real -> Real, t225_DT_adc0_nco_freq=0, t225_DT_adc0_nco_phase=0, t225_DT_adc0_coarse_freq=0, t225_DT_adc0_nyquist_zone=Zone 1, t225_DT_adc0_cal_mode=Mode 2, t225_DT_adc1_enable=on, t225_DT_adc1_digital_output=Real, t225_DT_adc1_dec_mode=1x, t225_DT_adc1_sample_per_cycle=8, t225_DT_adc1_req_axis_clk=200, t225_DT_adc1_mixer_type=Bypassed, t225_DT_adc1_mixer_mode=Real -> Real, t225_DT_adc1_nco_freq=0, t225_DT_adc1_nco_phase=0, t225_DT_adc1_coarse_freq=0, t225_DT_adc1_nyquist_zone=Zone 1, t225_DT_adc1_cal_mode=Mode 2, Tile226_enable=on, t226_enable_mts=off, t226_sample_rate=1600, t226_clk_out=100, t226_enable_pll=on, t226_ref_clk=400, t226_axi_stream_clk=200, t226_QT_adc0_enable=on, t226_QT_adc0_digital_output=Real, t226_QT_adc0_dec_mode=1x, t226_QT_adc0_sample_per_cycle=8, t226_QT_adc0_req_axis_clk=250, t226_QT_adc0_mixer_type=Bypassed, t226_QT_adc0_mixer_mode=Real -> Real, t226_QT_adc0_nco_freq=0, t226_QT_adc0_nco_phase=0, t226_QT_adc0_coarse_freq=0, t226_QT_adc0_nyquist_zone=Zone 1, t226_QT_adc0_cal_mode=Mode 2, t226_QT_adc1_enable=off, t226_QT_adc1_digital_output=Real, t226_QT_adc1_dec_mode=1x, t226_QT_adc1_sample_per_cycle=8, t226_QT_adc1_req_axis_clk=250, t226_QT_adc1_mixer_type=Bypassed, t226_QT_adc1_mixer_mode=Real -> Real, t226_QT_adc1_nco_freq=0, t226_QT_adc1_nco_phase=0, t226_QT_adc1_coarse_freq=0, t226_QT_adc1_nyquist_zone=Zone 1, t226_QT_adc1_cal_mode=Mode 2, t226_QT_adc2_enable=off, t226_QT_adc2_digital_output=Real, t226_QT_adc2_dec_mode=1x, t226_QT_adc2_sample_per_cycle=8, t226_QT_adc2_req_axis_clk=250, t226_QT_adc2_mixer_type=Bypassed, t226_QT_adc2_mixer_mode=Real -> Real, t226_QT_adc2_nco_freq=0, t226_QT_adc2_nco_phase=0, t226_QT_adc2_coarse_freq=0, t226_QT_adc2_nyquist_zone=Zone 1, t226_QT_adc2_cal_mode=Mode 2, t226_QT_adc3_enable=off, t226_QT_adc3_digital_output=Real, t226_QT_adc3_dec_mode=1x, t226_QT_adc3_sample_per_cycle=8, t226_QT_adc3_req_axis_clk=250, t226_QT_adc3_mixer_type=Bypassed, t226_QT_adc3_mixer_mode=Real -> Real, t226_QT_adc3_nco_freq=0, t226_QT_adc3_nco_phase=0, t226_QT_adc3_coarse_freq=0, t226_QT_adc3_nyquist_zone=Zone 1, t226_QT_adc3_cal_mode=Mode 2, t226_DT_adc0_enable=on, t226_DT_adc0_digital_output=Real, t226_DT_adc0_dec_mode=1x, t226_DT_adc0_sample_per_cycle=8, t226_DT_adc0_req_axis_clk=200, t226_DT_adc0_mixer_type=Bypassed, t226_DT_adc0_mixer_mode=Real -> Real, t226_DT_adc0_nco_freq=0, t226_DT_adc0_nco_phase=0, t226_DT_adc0_coarse_freq=0, t226_DT_adc0_nyquist_zone=Zone 1, t226_DT_adc0_cal_mode=Mode 2, t226_DT_adc1_enable=on, t226_DT_adc1_digital_output=Real, t226_DT_adc1_dec_mode=1x, t226_DT_adc1_sample_per_cycle=8, t226_DT_adc1_req_axis_clk=200, t226_DT_adc1_mixer_type=Bypassed, t226_DT_adc1_mixer_mode=Real -> Real, t226_DT_adc1_nco_freq=0, t226_DT_adc1_nco_phase=0, t226_DT_adc1_coarse_freq=0, t226_DT_adc1_nyquist_zone=Zone 1, t226_DT_adc1_cal_mode=Mode 2, Tile227_enable=on, t227_enable_mts=off, t227_sample_rate=1600, t227_clk_out=100, t227_enable_pll=on, t227_ref_clk=400, t227_axi_stream_clk=200, t227_QT_adc0_enable=on, t227_QT_adc0_digital_output=Real, t227_QT_adc0_dec_mode=1x, t227_QT_adc0_sample_per_cycle=8, t227_QT_adc0_req_axis_clk=250, t227_QT_adc0_mixer_type=Bypassed, t227_QT_adc0_mixer_mode=Real -> Real, t227_QT_adc0_nco_freq=0, t227_QT_adc0_nco_phase=0, t227_QT_adc0_coarse_freq=0, t227_QT_adc0_nyquist_zone=Zone 1, t227_QT_adc0_cal_mode=Mode 2, t227_QT_adc1_enable=off, t227_QT_adc1_digital_output=Real, t227_QT_adc1_dec_mode=1x, t227_QT_adc1_sample_per_cycle=8, t227_QT_adc1_req_axis_clk=250, t227_QT_adc1_mixer_type=Bypassed, t227_QT_adc1_mixer_mode=Real -> Real, t227_QT_adc1_nco_freq=0, t227_QT_adc1_nco_phase=0, t227_QT_adc1_coarse_freq=0, t227_QT_adc1_nyquist_zone=Zone 1, t227_QT_adc1_cal_mode=Mode 2, t227_QT_adc2_enable=off, t227_QT_adc2_digital_output=Real, t227_QT_adc2_dec_mode=1x, t227_QT_adc2_sample_per_cycle=8, t227_QT_adc2_req_axis_clk=250, t227_QT_adc2_mixer_type=Bypassed, t227_QT_adc2_mixer_mode=Real -> Real, t227_QT_adc2_nco_freq=0, t227_QT_adc2_nco_phase=0, t227_QT_adc2_coarse_freq=0, t227_QT_adc2_nyquist_zone=Zone 1, t227_QT_adc2_cal_mode=Mode 2, t227_QT_adc3_enable=off, t227_QT_adc3_digital_output=Real, t227_QT_adc3_dec_mode=1x, t227_QT_adc3_sample_per_cycle=8, t227_QT_adc3_req_axis_clk=250, t227_QT_adc3_mixer_type=Bypassed, t227_QT_adc3_mixer_mode=Real -> Real, t227_QT_adc3_nco_freq=0, t227_QT_adc3_nco_phase=0, t227_QT_adc3_coarse_freq=0, t227_QT_adc3_nyquist_zone=Zone 1, t227_QT_adc3_cal_mode=Mode 2, t227_DT_adc0_enable=on, t227_DT_adc0_digital_output=Real, t227_DT_adc0_dec_mode=1x, t227_DT_adc0_sample_per_cycle=8, t227_DT_adc0_req_axis_clk=200, t227_DT_adc0_mixer_type=Bypassed, t227_DT_adc0_mixer_mode=Real -> Real, t227_DT_adc0_nco_freq=0, t227_DT_adc0_nco_phase=0, t227_DT_adc0_coarse_freq=0, t227_DT_adc0_nyquist_zone=Zone 1, t227_DT_adc0_cal_mode=Mode 2, t227_DT_adc1_enable=on, t227_DT_adc1_digital_output=Real, t227_DT_adc1_dec_mode=1x, t227_DT_adc1_sample_per_cycle=8, t227_DT_adc1_req_axis_clk=200, t227_DT_adc1_mixer_type=Bypassed, t227_DT_adc1_mixer_mode=Real -> Real, t227_DT_adc1_nco_freq=0, t227_DT_adc1_nco_phase=0, t227_DT_adc1_coarse_freq=0, t227_DT_adc1_nyquist_zone=Zone 1, t227_DT_adc1_cal_mode=Mode 2, Tile228_enable=off, t228_enable_mts=off, t228_sample_rate=2000.0, t228_clk_out=125, t228_enable_pll=off, t228_ref_clk=2000, t228_axi_stream_clk=[], t228_output_power=20, t228_QT_dac0_enable=on, t228_QT_dac0_analog_output=Real, t228_QT_dac0_inter_mode=1x, t228_QT_dac0_sample_per_cycle=8, t228_QT_dac0_req_axis_clk=250, t228_QT_dac0_datapath_mode=DUC 0 to Fs/2, t228_QT_dac0_mixer_type=Coarse, t228_QT_dac0_mixer_mode=Real -> Real, t228_QT_dac0_nco_freq=0, t228_QT_dac0_nco_phase=0, t228_QT_dac0_coarse_freq=0, t228_QT_dac0_nyquist_zone=Zone 1, t228_QT_dac0_decode_mode=SNR Optimized, t228_QT_dac1_enable=off, t228_QT_dac1_analog_output=Real, t228_QT_dac1_inter_mode=1x, t228_QT_dac1_sample_per_cycle=8, t228_QT_dac1_req_axis_clk=250, t228_QT_dac1_datapath_mode=DUC 0 to Fs/2, t228_QT_dac1_mixer_type=Coarse, t228_QT_dac1_mixer_mode=Real -> Real, t228_QT_dac1_nco_freq=0, t228_QT_dac1_nco_phase=0, t228_QT_dac1_coarse_freq=0, t228_QT_dac1_nyquist_zone=Zone 1, t228_QT_dac1_decode_mode=SNR Optimized, t228_QT_dac2_enable=off, t228_QT_dac2_analog_output=Real, t228_QT_dac2_inter_mode=1x, t228_QT_dac2_sample_per_cycle=8, t228_QT_dac2_req_axis_clk=250, t228_QT_dac2_datapath_mode=DUC 0 to Fs/2, t228_QT_dac2_mixer_type=Coarse, t228_QT_dac2_mixer_mode=Real -> Real, t228_QT_dac2_nco_freq=0, t228_QT_dac2_nco_phase=0, t228_QT_dac2_coarse_freq=0, t228_QT_dac2_nyquist_zone=Zone 1, t228_QT_dac2_decode_mode=SNR Optimized, t228_QT_dac3_enable=off, t228_QT_dac3_analog_output=Real, t228_QT_dac3_inter_mode=1x, t228_QT_dac3_sample_per_cycle=8, t228_QT_dac3_req_axis_clk=250, t228_QT_dac3_datapath_mode=DUC 0 to Fs/2, t228_QT_dac3_mixer_type=Coarse, t228_QT_dac3_mixer_mode=Real -> Real, t228_QT_dac3_nco_freq=0, t228_QT_dac3_nco_phase=0, t228_QT_dac3_coarse_freq=0, t228_QT_dac3_nyquist_zone=Zone 1, t228_QT_dac3_decode_mode=SNR Optimized, t228_DT_dac0_enable=off, t228_DT_dac0_analog_output=Real, t228_DT_dac0_inter_mode=1x, t228_DT_dac0_sample_per_cycle=8, t228_DT_dac0_req_axis_clk=250, t228_DT_dac0_mixer_type=Coarse, t228_DT_dac0_mixer_mode=Real -> Real, t228_DT_dac0_nco_freq=0, t228_DT_dac0_nco_phase=0, t228_DT_dac0_coarse_freq=0, t228_DT_dac0_nyquist_zone=Zone 1, t228_DT_dac0_decode_mode=SNR Optimized, t228_DT_dac1_enable=off, t228_DT_dac1_analog_output=Real, t228_DT_dac1_inter_mode=1x, t228_DT_dac1_sample_per_cycle=8, t228_DT_dac1_req_axis_clk=250, t228_DT_dac1_mixer_type=Coarse, t228_DT_dac1_mixer_mode=Real -> Real, t228_DT_dac1_nco_freq=0, t228_DT_dac1_nco_phase=0, t228_DT_dac1_coarse_freq=0, t228_DT_dac1_nyquist_zone=Zone 1, t228_DT_dac1_decode_mode=SNR Optimized, Tile229_enable=off, t229_enable_mts=off, t229_sample_rate=2000.0, t229_clk_out=125, t229_enable_pll=off, t229_ref_clk=2000, t229_axi_stream_clk=[], t229_output_power=20, t229_QT_dac0_enable=on, t229_QT_dac0_analog_output=Real, t229_QT_dac0_inter_mode=1x, t229_QT_dac0_sample_per_cycle=8, t229_QT_dac0_req_axis_clk=250, t229_QT_dac0_datapath_mode=DUC 0 to Fs/2, t229_QT_dac0_mixer_type=Coarse, t229_QT_dac0_mixer_mode=Real -> Real, t229_QT_dac0_nco_freq=0, t229_QT_dac0_nco_phase=0, t229_QT_dac0_coarse_freq=0, t229_QT_dac0_nyquist_zone=Zone 1, t229_QT_dac0_decode_mode=SNR Optimized, t229_QT_dac1_enable=off, t229_QT_dac1_analog_output=Real, t229_QT_dac1_inter_mode=1x, t229_QT_dac1_sample_per_cycle=8, t229_QT_dac1_req_axis_clk=250, t229_QT_dac1_datapath_mode=DUC 0 to Fs/2, t229_QT_dac1_mixer_type=Coarse, t229_QT_dac1_mixer_mode=Real -> Real, t229_QT_dac1_nco_freq=0, t229_QT_dac1_nco_phase=0, t229_QT_dac1_coarse_freq=0, t229_QT_dac1_nyquist_zone=Zone 1, t229_QT_dac1_decode_mode=SNR Optimized, t229_QT_dac2_enable=off, t229_QT_dac2_analog_output=Real, t229_QT_dac2_inter_mode=1x, t229_QT_dac2_sample_per_cycle=8, t229_QT_dac2_req_axis_clk=250, t229_QT_dac2_datapath_mode=DUC 0 to Fs/2, t229_QT_dac2_mixer_type=Coarse, t229_QT_dac2_mixer_mode=Real -> Real, t229_QT_dac2_nco_freq=0, t229_QT_dac2_nco_phase=0, t229_QT_dac2_coarse_freq=0, t229_QT_dac2_nyquist_zone=Zone 1, t229_QT_dac2_decode_mode=SNR Optimized, t229_QT_dac3_enable=off, t229_QT_dac3_analog_output=Real, t229_QT_dac3_inter_mode=1x, t229_QT_dac3_sample_per_cycle=8, t229_QT_dac3_req_axis_clk=250, t229_QT_dac3_datapath_mode=DUC 0 to Fs/2, t229_QT_dac3_mixer_type=Coarse, t229_QT_dac3_mixer_mode=Real -> Real, t229_QT_dac3_nco_freq=0, t229_QT_dac3_nco_phase=0, t229_QT_dac3_coarse_freq=0, t229_QT_dac3_nyquist_zone=Zone 1, t229_QT_dac3_decode_mode=SNR Optimized, t229_DT_dac0_enable=off, t229_DT_dac0_analog_output=Real, t229_DT_dac0_inter_mode=1x, t229_DT_dac0_sample_per_cycle=8, t229_DT_dac0_req_axis_clk=250, t229_DT_dac0_mixer_type=Coarse, t229_DT_dac0_mixer_mode=Real -> Real, t229_DT_dac0_nco_freq=0, t229_DT_dac0_nco_phase=0, t229_DT_dac0_coarse_freq=0, t229_DT_dac0_nyquist_zone=Zone 1, t229_DT_dac0_decode_mode=SNR Optimized, t229_DT_dac1_enable=off, t229_DT_dac1_analog_output=Real, t229_DT_dac1_inter_mode=1x, t229_DT_dac1_sample_per_cycle=8, t229_DT_dac1_req_axis_clk=250, t229_DT_dac1_mixer_type=Coarse, t229_DT_dac1_mixer_mode=Real -> Real, t229_DT_dac1_nco_freq=0, t229_DT_dac1_nco_phase=0, t229_DT_dac1_coarse_freq=0, t229_DT_dac1_nyquist_zone=Zone 1, t229_DT_dac1_decode_mode=SNR Optimized, Tile230_enable=off, t230_enable_mts=off, t230_sample_rate=2000.0, t230_clk_out=125, t230_enable_pll=off, t230_ref_clk=2000, t230_axi_stream_clk=[], t230_output_power=20, t230_QT_dac0_enable=on, t230_QT_dac0_analog_output=Real, t230_QT_dac0_inter_mode=1x, t230_QT_dac0_sample_per_cycle=8, t230_QT_dac0_req_axis_clk=250, t230_QT_dac0_datapath_mode=DUC 0 to Fs/2, t230_QT_dac0_mixer_type=Coarse, t230_QT_dac0_mixer_mode=Real -> Real, t230_QT_dac0_nco_freq=0, t230_QT_dac0_nco_phase=0, t230_QT_dac0_coarse_freq=0, t230_QT_dac0_nyquist_zone=Zone 1, t230_QT_dac0_decode_mode=SNR Optimized, t230_QT_dac1_enable=off, t230_QT_dac1_analog_output=Real, t230_QT_dac1_inter_mode=1x, t230_QT_dac1_sample_per_cycle=8, t230_QT_dac1_req_axis_clk=250, t230_QT_dac1_datapath_mode=DUC 0 to Fs/2, t230_QT_dac1_mixer_type=Coarse, t230_QT_dac1_mixer_mode=Real -> Real, t230_QT_dac1_nco_freq=0, t230_QT_dac1_nco_phase=0, t230_QT_dac1_coarse_freq=0, t230_QT_dac1_nyquist_zone=Zone 1, t230_QT_dac1_decode_mode=SNR Optimized, t230_QT_dac2_enable=off, t230_QT_dac2_analog_output=Real, t230_QT_dac2_inter_mode=1x, t230_QT_dac2_sample_per_cycle=8, t230_QT_dac2_req_axis_clk=250, t230_QT_dac2_datapath_mode=DUC 0 to Fs/2, t230_QT_dac2_mixer_type=Coarse, t230_QT_dac2_mixer_mode=Real -> Real, t230_QT_dac2_nco_freq=0, t230_QT_dac2_nco_phase=0, t230_QT_dac2_coarse_freq=0, t230_QT_dac2_nyquist_zone=Zone 1, t230_QT_dac2_decode_mode=SNR Optimized, t230_QT_dac3_enable=off, t230_QT_dac3_analog_output=Real, t230_QT_dac3_inter_mode=1x, t230_QT_dac3_sample_per_cycle=8, t230_QT_dac3_req_axis_clk=250, t230_QT_dac3_datapath_mode=DUC 0 to Fs/2, t230_QT_dac3_mixer_type=Coarse, t230_QT_dac3_mixer_mode=Real -> Real, t230_QT_dac3_nco_freq=0, t230_QT_dac3_nco_phase=0, t230_QT_dac3_coarse_freq=0, t230_QT_dac3_nyquist_zone=Zone 1, t230_QT_dac3_decode_mode=SNR Optimized, t230_DT_dac0_enable=off, t230_DT_dac0_analog_output=Real, t230_DT_dac0_inter_mode=1x, t230_DT_dac0_sample_per_cycle=8, t230_DT_dac0_req_axis_clk=250, t230_DT_dac0_mixer_type=Coarse, t230_DT_dac0_mixer_mode=Real -> Real, t230_DT_dac0_nco_freq=0, t230_DT_dac0_nco_phase=0, t230_DT_dac0_coarse_freq=0, t230_DT_dac0_nyquist_zone=Zone 1, t230_DT_dac0_decode_mode=SNR Optimized, t230_DT_dac1_enable=off, t230_DT_dac1_analog_output=Real, t230_DT_dac1_inter_mode=1x, t230_DT_dac1_sample_per_cycle=8, t230_DT_dac1_req_axis_clk=250, t230_DT_dac1_mixer_type=Coarse, t230_DT_dac1_mixer_mode=Real -> Real, t230_DT_dac1_nco_freq=0, t230_DT_dac1_nco_phase=0, t230_DT_dac1_coarse_freq=0, t230_DT_dac1_nyquist_zone=Zone 1, t230_DT_dac1_decode_mode=SNR Optimized, Tile231_enable=off, t231_enable_mts=off, t231_sample_rate=2000.0, t231_clk_out=125, t231_enable_pll=off, t231_ref_clk=2000, t231_axi_stream_clk=[], t231_output_power=20, t231_QT_dac0_enable=on, t231_QT_dac0_analog_output=Real, t231_QT_dac0_inter_mode=1x, t231_QT_dac0_sample_per_cycle=8, t231_QT_dac0_req_axis_clk=250, t231_QT_dac0_datapath_mode=DUC 0 to Fs/2, t231_QT_dac0_mixer_type=Coarse, t231_QT_dac0_mixer_mode=Real -> Real, t231_QT_dac0_nco_freq=0, t231_QT_dac0_nco_phase=0, t231_QT_dac0_coarse_freq=0, t231_QT_dac0_nyquist_zone=Zone 1, t231_QT_dac0_decode_mode=SNR Optimized, t231_QT_dac1_enable=off, t231_QT_dac1_analog_output=Real, t231_QT_dac1_inter_mode=1x, t231_QT_dac1_sample_per_cycle=8, t231_QT_dac1_req_axis_clk=250, t231_QT_dac1_datapath_mode=DUC 0 to Fs/2, t231_QT_dac1_mixer_type=Coarse, t231_QT_dac1_mixer_mode=Real -> Real, t231_QT_dac1_nco_freq=0, t231_QT_dac1_nco_phase=0, t231_QT_dac1_coarse_freq=0, t231_QT_dac1_nyquist_zone=Zone 1, t231_QT_dac1_decode_mode=SNR Optimized, t231_QT_dac2_enable=off, t231_QT_dac2_analog_output=Real, t231_QT_dac2_inter_mode=1x, t231_QT_dac2_sample_per_cycle=8, t231_QT_dac2_req_axis_clk=250, t231_QT_dac2_datapath_mode=DUC 0 to Fs/2, t231_QT_dac2_mixer_type=Coarse, t231_QT_dac2_mixer_mode=Real -> Real, t231_QT_dac2_nco_freq=0, t231_QT_dac2_nco_phase=0, t231_QT_dac2_coarse_freq=0, t231_QT_dac2_nyquist_zone=Zone 1, t231_QT_dac2_decode_mode=SNR Optimized, t231_QT_dac3_enable=off, t231_QT_dac3_analog_output=Real, t231_QT_dac3_inter_mode=1x, t231_QT_dac3_sample_per_cycle=8, t231_QT_dac3_req_axis_clk=250, t231_QT_dac3_datapath_mode=DUC 0 to Fs/2, t231_QT_dac3_mixer_type=Coarse, t231_QT_dac3_mixer_mode=Real -> Real, t231_QT_dac3_nco_freq=0, t231_QT_dac3_nco_phase=0, t231_QT_dac3_coarse_freq=0, t231_QT_dac3_nyquist_zone=Zone 1, t231_QT_dac3_decode_mode=SNR Optimized, t231_DT_dac0_enable=off, t231_DT_dac0_analog_output=Real, t231_DT_dac0_inter_mode=1x, t231_DT_dac0_sample_per_cycle=8, t231_DT_dac0_req_axis_clk=250, t231_DT_dac0_mixer_type=Coarse, t231_DT_dac0_mixer_mode=Real -> Real, t231_DT_dac0_nco_freq=0, t231_DT_dac0_nco_phase=0, t231_DT_dac0_coarse_freq=0, t231_DT_dac0_nyquist_zone=Zone 1, t231_DT_dac0_decode_mode=SNR Optimized, t231_DT_dac1_enable=off, t231_DT_dac1_analog_output=Real, t231_DT_dac1_inter_mode=1x, t231_DT_dac1_sample_per_cycle=8, t231_DT_dac1_req_axis_clk=250, t231_DT_dac1_mixer_type=Coarse, t231_DT_dac1_mixer_mode=Real -> Real, t231_DT_dac1_nco_freq=0, t231_DT_dac1_nco_phase=0, t231_DT_dac1_coarse_freq=0, t231_DT_dac1_nyquist_zone=Zone 1, t231_DT_dac1_decode_mode=SNR Optimized, t224_has_adc_clk=on, t224_adc_clk_src=224, t224_clk_dist=Input Refclk, t225_has_adc_clk=off, t225_adc_clk_src=224, t225_clk_dist=None, t226_has_adc_clk=on, t226_adc_clk_src=226, t226_clk_dist=Input Refclk, t227_has_adc_clk=off, t227_adc_clk_src=226, t227_clk_dist=None, t228_has_dac_clk=on, t228_dac_clk_src=228, t228_clk_dist=Input Refclk, t229_has_dac_clk=off, t229_dac_clk_src=228, t229_clk_dist=None, t230_has_dac_clk=on, t230_dac_clk_src=230, t230_clk_dist=Input Refclk, t231_has_dac_clk=off, t231_dac_clk_src=230, t231_clk_dist=None, maskdoneopening=0}
      mask prompts: Tile224_enable "Enable Tile"; t224_enable_mts "Enable Multi-Tile Sync"; t224_sample_rate "Sampling Rate (Msps)"; t224_clk_out "Clock Out (MHz)"; t224_enable_pll "Enable Tile PLLs"; t224_ref_clk "Reference Clock (MHz)"; t224_axi_stream_clk "Required AXI4-Stream Clock (MHz)"; t224_QT_adc0_enable "Enable ADC"; t224_QT_adc0_digital_output "Digital Output Data"; t224_QT_adc0_dec_mode "Decimation Mode"; t224_QT_adc0_sample_per_cycle "Samples per AXI4-Stream Cycle"; t224_QT_adc0_mixer_type "Mixer Type"; t224_QT_adc0_mixer_mode "Mixer Mode"; t224_QT_adc0_nco_freq "NCO Frequency (GHz)"; t224_QT_adc0_nco_phase "NCO Phase"; t224_QT_adc0_coarse_freq "Frequency"; t224_QT_adc0_nyquist_zone "Nyquist Zone"; t224_QT_adc0_cal_mode "Calibration Mode"; t224_QT_adc1_enable "Enable ADC"; t224_QT_adc1_digital_output "Digital Output Data"; t224_QT_adc1_dec_mode "Decimation Mode"; t224_QT_adc1_sample_per_cycle "Samples per AXI4-Stream Cycle"; t224_QT_adc1_mixer_type "Mixer Type"; t224_QT_adc1_mixer_mode "Mixer Mode"; t224_QT_adc1_nco_freq "NCO Frequency (GHz)"; t224_QT_adc1_nco_phase "NCO Phase"; t224_QT_adc1_coarse_freq "Frequency"; t224_QT_adc1_nyquist_zone "Nyquist Zone"; t224_QT_adc1_cal_mode "Calibration Mode"; t224_QT_adc2_enable "Enable ADC"; t224_QT_adc2_digital_output "Digital Output Data"; t224_QT_adc2_dec_mode "Decimation Mode"; t224_QT_adc2_sample_per_cycle "Samples per AXI4-Stream Cycle"; t224_QT_adc2_mixer_type "Mixer Type"; t224_QT_adc2_mixer_mode "Mixer Mode"; t224_QT_adc2_nco_freq "NCO Frequency (GHz)"; t224_QT_adc2_nco_phase "NCO Phase"; t224_QT_adc2_coarse_freq "Frequency"; t224_QT_adc2_nyquist_zone "Nyquist Zone"; t224_QT_adc2_cal_mode "Calibration Mode"; t224_QT_adc3_enable "Enable ADC"; t224_QT_adc3_digital_output "Digital Output Data"; t224_QT_adc3_dec_mode "Decimation Mode"; t224_QT_adc3_sample_per_cycle "Samples per AXI4-Stream Cycle"; t224_QT_adc3_mixer_type "Mixer Type"; t224_QT_adc3_mixer_mode "Mixer Mode"; t224_QT_adc3_nco_freq "NCO Frequency (GHz)"; t224_QT_adc3_nco_phase "NCO Phase"; t224_QT_adc3_coarse_freq "Frequency"; t224_QT_adc3_nyquist_zone "Nyquist Zone"; t224_QT_adc3_cal_mode "Calibration Mode"; t224_DT_adc0_enable "Enable ADC"; t224_DT_adc0_digital_output "Digital Output Data"; t224_DT_adc0_dec_mode "Decimation Mode"; t224_DT_adc0_sample_per_cycle "Samples per AXI4-Stream Cycle"; t224_DT_adc0_mixer_type "Mixer Type"; t224_DT_adc0_mixer_mode "Mixer Mode"; t224_DT_adc0_nco_freq "NCO Frequency (GHz)"; t224_DT_adc0_nco_phase "NCO Phase"; t224_DT_adc0_coarse_freq "Frequency"; t224_DT_adc0_nyquist_zone "Nyquist Zone"; t224_DT_adc0_cal_mode "Calibration Mode"; t224_DT_adc1_enable "Enable ADC"; t224_DT_adc1_digital_output "Digital Output Data"; t224_DT_adc1_dec_mode "Decimation Mode"; t224_DT_adc1_sample_per_cycle "Samples per AXI4-Stream Cycle"; t224_DT_adc1_mixer_type "Mixer Type"; t224_DT_adc1_mixer_mode "Mixer Mode"; t224_DT_adc1_nco_freq "NCO Frequency (GHz)"; t224_DT_adc1_nco_phase "NCO Phase"; t224_DT_adc1_coarse_freq "Frequency"; t224_DT_adc1_nyquist_zone "Nyquist Zone"; t224_DT_adc1_cal_mode "Calibration Mode"; Tile225_enable "Enable Tile"; t225_enable_mts "Enable Multi-Tile Sync"; t225_sample_rate "Sampling Rate (Msps)"; t225_clk_out "Clock Out (MHz)"; t225_enable_pll "Enable Tile PLLs"; t225_ref_clk "Reference Clock (MHz)"; t225_axi_stream_clk "Required AXI4-Stream Clock (MHz)"; t225_QT_adc0_enable "Enable ADC"; t225_QT_adc0_digital_output "Digital Output Data"; t225_QT_adc0_dec_mode "Decimation Mode"; t225_QT_adc0_sample_per_cycle "Samples per AXI4-Stream Cycle"; t225_QT_adc0_mixer_type "Mixer Type"; t225_QT_adc0_mixer_mode "Mixer Mode"; t225_QT_adc0_nco_freq "NCO Frequency (GHz)"; t225_QT_adc0_nco_phase "NCO Phase"; t225_QT_adc0_coarse_freq "Frequency"; t225_QT_adc0_nyquist_zone "Nyquist Zone"; t225_QT_adc0_cal_mode "Calibration Mode"; t225_QT_adc1_enable "Enable ADC"; t225_QT_adc1_digital_output "Digital Output Data"; t225_QT_adc1_dec_mode "Decimation Mode"; t225_QT_adc1_sample_per_cycle "Samples per AXI4-Stream Cycle"; t225_QT_adc1_mixer_type "Mixer Type"; t225_QT_adc1_mixer_mode "Mixer Mode"; t225_QT_adc1_nco_freq "NCO Frequency (GHz)"; t225_QT_adc1_nco_phase "NCO Phase"; t225_QT_adc1_coarse_freq "Frequency"; t225_QT_adc1_nyquist_zone "Nyquist Zone"; t225_QT_adc1_cal_mode "Calibration Mode"; t225_QT_adc2_enable "Enable ADC"; t225_QT_adc2_digital_output "Digital Output Data"; t225_QT_adc2_dec_mode "Decimation Mode"; t225_QT_adc2_sample_per_cycle "Samples per AXI4-Stream Cycle"; t225_QT_adc2_mixer_type "Mixer Type"; t225_QT_adc2_mixer_mode "Mixer Mode"; t225_QT_adc2_nco_freq "NCO Frequency (GHz)"; t225_QT_adc2_nco_phase "NCO Phase"; t225_QT_adc2_coarse_freq "Frequency"; t225_QT_adc2_nyquist_zone "Nyquist Zone"; t225_QT_adc2_cal_mode "Calibration Mode"; t225_QT_adc3_enable "Enable ADC"; t225_QT_adc3_digital_output "Digital Output Data"; t225_QT_adc3_dec_mode "Decimation Mode"; t225_QT_adc3_sample_per_cycle "Samples per AXI4-Stream Cycle"; t225_QT_adc3_mixer_type "Mixer Type"; t225_QT_adc3_mixer_mode "Mixer Mode"; t225_QT_adc3_nco_freq "NCO Frequency (GHz)"; t225_QT_adc3_nco_phase "NCO Phase"; t225_QT_adc3_coarse_freq "Frequency"; t225_QT_adc3_nyquist_zone "Nyquist Zone"; t225_QT_adc3_cal_mode "Calibration Mode"; t225_DT_adc0_enable "Enable ADC"; t225_DT_adc0_digital_output "Digital Output Data"; t225_DT_adc0_dec_mode "Decimation Mode"; t225_DT_adc0_sample_per_cycle "Samples per AXI4-Stream Cycle"; t225_DT_adc0_mixer_type "Mixer Type"; t225_DT_adc0_mixer_mode "Mixer Mode"; t225_DT_adc0_nco_freq "NCO Frequency (GHz)"; t225_DT_adc0_nco_phase "NCO Phase"; t225_DT_adc0_coarse_freq "Frequency"; t225_DT_adc0_nyquist_zone "Nyquist Zone"; t225_DT_adc0_cal_mode "Calibration Mode"; t225_DT_adc1_enable "Enable ADC"; t225_DT_adc1_digital_output "Digital Output Data"; t225_DT_adc1_dec_mode "Decimation Mode"; t225_DT_adc1_sample_per_cycle "Samples per AXI4-Stream Cycle"; t225_DT_adc1_mixer_type "Mixer Type"; t225_DT_adc1_mixer_mode "Mixer Mode"; t225_DT_adc1_nco_freq "NCO Frequency (GHz)"; t225_DT_adc1_nco_phase "NCO Phase"; t225_DT_adc1_coarse_freq "Frequency"; t225_DT_adc1_nyquist_zone "Nyquist Zone"; t225_DT_adc1_cal_mode "Calibration Mode"; Tile226_enable "Enable Tile"; t226_enable_mts "Enable Multi-Tile Sync"; t226_sample_rate "Sampling Rate (Msps)"; t226_clk_out "Clock Out (MHz)"; t226_enable_pll "Enable Tile PLLs"; t226_ref_clk "Reference Clock (MHz)"; t226_axi_stream_clk "Required AXI4-Stream Clock (MHz)"; t226_QT_adc0_enable "Enable ADC"; t226_QT_adc0_digital_output "Digital Output Data"; t226_QT_adc0_dec_mode "Decimation Mode"; t226_QT_adc0_sample_per_cycle "Samples per AXI4-Stream Cycle"; t226_QT_adc0_mixer_type "Mixer Type"; t226_QT_adc0_mixer_mode "Mixer Mode"; t226_QT_adc0_nco_freq "NCO Frequency (GHz)"; t226_QT_adc0_nco_phase "NCO Phase"; t226_QT_adc0_coarse_freq "Frequency"; t226_QT_adc0_nyquist_zone "Nyquist Zone"; t226_QT_adc0_cal_mode "Calibration Mode"; t226_QT_adc1_enable "Enable ADC"; t226_QT_adc1_digital_output "Digital Output Data"; t226_QT_adc1_dec_mode "Decimation Mode"; t226_QT_adc1_sample_per_cycle "Samples per AXI4-Stream Cycle"; t226_QT_adc1_mixer_type "Mixer Type"; t226_QT_adc1_mixer_mode "Mixer Mode"; t226_QT_adc1_nco_freq "NCO Frequency (GHz)"; t226_QT_adc1_nco_phase "NCO Phase"; t226_QT_adc1_coarse_freq "Frequency"; t226_QT_adc1_nyquist_zone "Nyquist Zone"; t226_QT_adc1_cal_mode "Calibration Mode"; t226_QT_adc2_enable "Enable ADC"; t226_QT_adc2_digital_output "Digital Output Data"; t226_QT_adc2_dec_mode "Decimation Mode"; t226_QT_adc2_sample_per_cycle "Samples per AXI4-Stream Cycle"; t226_QT_adc2_mixer_type "Mixer Type"; t226_QT_adc2_mixer_mode "Mixer Mode"; t226_QT_adc2_nco_freq "NCO Frequency (GHz)"; t226_QT_adc2_nco_phase "NCO Phase"; t226_QT_adc2_coarse_freq "Frequency"; t226_QT_adc2_nyquist_zone "Nyquist Zone"; t226_QT_adc2_cal_mode "Calibration Mode"; t226_QT_adc3_enable "Enable ADC"; t226_QT_adc3_digital_output "Digital Output Data"; t226_QT_adc3_dec_mode "Decimation Mode"; t226_QT_adc3_sample_per_cycle "Samples per AXI4-Stream Cycle"; t226_QT_adc3_mixer_type "Mixer Type"; t226_QT_adc3_mixer_mode "Mixer Mode"; t226_QT_adc3_nco_freq "NCO Frequency (GHz)"; t226_QT_adc3_nco_phase "NCO Phase"; t226_QT_adc3_coarse_freq "Frequency"; t226_QT_adc3_nyquist_zone "Nyquist Zone"; t226_QT_adc3_cal_mode "Calibration Mode"; t226_DT_adc0_enable "Enable ADC"; t226_DT_adc0_digital_output "Digital Output Data"; t226_DT_adc0_dec_mode "Decimation Mode"; t226_DT_adc0_sample_per_cycle "Samples per AXI4-Stream Cycle"; t226_DT_adc0_mixer_type "Mixer Type"; t226_DT_adc0_mixer_mode "Mixer Mode"; t226_DT_adc0_nco_freq "NCO Frequency (GHz)"; t226_DT_adc0_nco_phase "NCO Phase"; t226_DT_adc0_coarse_freq "Frequency"; t226_DT_adc0_nyquist_zone "Nyquist Zone"; t226_DT_adc0_cal_mode "Calibration Mode"; t226_DT_adc1_enable "Enable ADC"; t226_DT_adc1_digital_output "Digital Output Data"; t226_DT_adc1_dec_mode "Decimation Mode"; t226_DT_adc1_sample_per_cycle "Samples per AXI4-Stream Cycle"; t226_DT_adc1_mixer_type "Mixer Type"; t226_DT_adc1_mixer_mode "Mixer Mode"; t226_DT_adc1_nco_freq "NCO Frequency (GHz)"; t226_DT_adc1_nco_phase "NCO Phase"; t226_DT_adc1_coarse_freq "Frequency"; t226_DT_adc1_nyquist_zone "Nyquist Zone"; t226_DT_adc1_cal_mode "Calibration Mode"; Tile227_enable "Enable Tile"; t227_enable_mts "Enable Multi-Tile Sync"; t227_sample_rate "Sampling Rate (Msps)"; t227_clk_out "Clock Out (MHz)"; t227_enable_pll "Enable Tile PLLs"; t227_ref_clk "Reference Clock (MHz)"; t227_axi_stream_clk "Required AXI4-Stream Clock (MHz)"; t227_QT_adc0_enable "Enable ADC"; t227_QT_adc0_digital_output "Digital Output Data"; t227_QT_adc0_dec_mode "Decimation Mode"; t227_QT_adc0_sample_per_cycle "Samples per AXI4-Stream Cycle"; t227_QT_adc0_mixer_type "Mixer Type"; t227_QT_adc0_mixer_mode "Mixer Mode"; t227_QT_adc0_nco_freq "NCO Frequency (GHz)"; t227_QT_adc0_nco_phase "NCO Phase"; t227_QT_adc0_coarse_freq "Frequency"; t227_QT_adc0_nyquist_zone "Nyquist Zone"; t227_QT_adc0_cal_mode "Calibration Mode"; t227_QT_adc1_enable "Enable ADC"; t227_QT_adc1_digital_output "Digital Output Data"; t227_QT_adc1_dec_mode "Decimation Mode"; t227_QT_adc1_sample_per_cycle "Samples per AXI4-Stream Cycle"; t227_QT_adc1_mixer_type "Mixer Type"; t227_QT_adc1_mixer_mode "Mixer Mode"; t227_QT_adc1_nco_freq "NCO Frequency (GHz)"; t227_QT_adc1_nco_phase "NCO Phase"; t227_QT_adc1_coarse_freq "Frequency"; t227_QT_adc1_nyquist_zone "Nyquist Zone"; t227_QT_adc1_cal_mode "Calibration Mode"; t227_QT_adc2_enable "Enable ADC"; t227_QT_adc2_digital_output "Digital Output Data"; t227_QT_adc2_dec_mode "Decimation Mode"; t227_QT_adc2_sample_per_cycle "Samples per AXI4-Stream Cycle"; t227_QT_adc2_mixer_type "Mixer Type"; t227_QT_adc2_mixer_mode "Mixer Mode"; t227_QT_adc2_nco_freq "NCO Frequency (GHz)"; t227_QT_adc2_nco_phase "NCO Phase"; t227_QT_adc2_coarse_freq "Frequency"; t227_QT_adc2_nyquist_zone "Nyquist Zone"; t227_QT_adc2_cal_mode "Calibration Mode"; t227_QT_adc3_enable "Enable ADC"; t227_QT_adc3_digital_output "Digital Output Data"; t227_QT_adc3_dec_mode "Decimation Mode"; t227_QT_adc3_sample_per_cycle "Samples per AXI4-Stream Cycle"; t227_QT_adc3_mixer_type "Mixer Type"; t227_QT_adc3_mixer_mode "Mixer Mode"; t227_QT_adc3_nco_freq "NCO Frequency (GHz)"; t227_QT_adc3_nco_phase "NCO Phase"; t227_QT_adc3_coarse_freq "Frequency"; t227_QT_adc3_nyquist_zone "Nyquist Zone"; t227_QT_adc3_cal_mode "Calibration Mode"; t227_DT_adc0_enable "Enable ADC"; t227_DT_adc0_digital_output "Digital Output Data"; t227_DT_adc0_dec_mode "Decimation Mode"; t227_DT_adc0_sample_per_cycle "Samples per AXI4-Stream Cycle"; t227_DT_adc0_mixer_type "Mixer Type"; t227_DT_adc0_mixer_mode "Mixer Mode"; t227_DT_adc0_nco_freq "NCO Frequency (GHz)"; t227_DT_adc0_nco_phase "NCO Phase"; t227_DT_adc0_coarse_freq "Frequency"; t227_DT_adc0_nyquist_zone "Nyquist Zone"; t227_DT_adc0_cal_mode "Calibration Mode"; t227_DT_adc1_enable "Enable ADC"; t227_DT_adc1_digital_output "Digital Output Data"; t227_DT_adc1_dec_mode "Decimation Mode"; t227_DT_adc1_sample_per_cycle "Samples per AXI4-Stream Cycle"; t227_DT_adc1_mixer_type "Mixer Type"; t227_DT_adc1_mixer_mode "Mixer Mode"; t227_DT_adc1_nco_freq "NCO Frequency (GHz)"; t227_DT_adc1_nco_phase "NCO Phase"; t227_DT_adc1_coarse_freq "Frequency"; t227_DT_adc1_nyquist_zone "Nyquist Zone"; t227_DT_adc1_cal_mode "Calibration Mode"; Tile228_enable "Enable Tile"; t228_enable_mts "Enable Multi-Tile Sync"; t228_sample_rate "Sampling Rate (Msps)"; t228_clk_out "Clock Out (MHz)"; t228_enable_pll "Enable Tile PLLs"; t228_ref_clk "Reference Clock (MHz)"; t228_axi_stream_clk "Required AXI4-Stream Clock (MHz)"; t228_output_power "Output Power"; t228_QT_dac0_enable "Enable DAC"; t228_QT_dac0_analog_output "Analog Output Data"; t228_QT_dac0_inter_mode "Interpolation Mode"; t228_QT_dac0_sample_per_cycle "Samples per AXI4-Stream Cycle"; t228_QT_dac0_datapath_mode "Datapath Mode"; t228_QT_dac0_mixer_type "Mixer Type"; t228_QT_dac0_mixer_mode "Mixer Mode"; t228_QT_dac0_nco_freq "NCO Frequency (GHz)"; t228_QT_dac0_nco_phase "NCO Phase"; t228_QT_dac0_coarse_freq "Frequency"; t228_QT_dac0_nyquist_zone "Nyquist Zone"; t228_QT_dac0_decode_mode "Decoder Mode"; t228_QT_dac1_enable "Enable DAC"; t228_QT_dac1_analog_output "Analog Output Data"; t228_QT_dac1_inter_mode "Interpolation Mode"; t228_QT_dac1_sample_per_cycle "Samples per AXI4-Stream Cycle"; t228_QT_dac1_datapath_mode "Datapath Mode"; t228_QT_dac1_mixer_type "Mixer Type"; t228_QT_dac1_mixer_mode "Mixer Mode"; t228_QT_dac1_nco_freq "NCO Frequency (GHz)"; t228_QT_dac1_nco_phase "NCO Phase"; t228_QT_dac1_coarse_freq "Frequency"; t228_QT_dac1_nyquist_zone "Nyquist Zone"; t228_QT_dac1_decode_mode "Decoder Mode"; t228_QT_dac2_enable "Enable DAC"; t228_QT_dac2_analog_output "Analog Output Data"; t228_QT_dac2_inter_mode "Interpolation Mode"; t228_QT_dac2_sample_per_cycle "Samples per AXI4-Stream Cycle"; t228_QT_dac2_datapath_mode "Datapath Mode"; t228_QT_dac2_mixer_type "Mixer Type"; t228_QT_dac2_mixer_mode "Mixer Mode"; t228_QT_dac2_nco_freq "NCO Frequency (GHz)"; t228_QT_dac2_nco_phase "NCO Phase"; t228_QT_dac2_coarse_freq "Frequency"; t228_QT_dac2_nyquist_zone "Nyquist Zone"; t228_QT_dac2_decode_mode "Decoder Mode"; t228_QT_dac3_enable "Enable DAC"; t228_QT_dac3_analog_output "Analog Output Data"; t228_QT_dac3_inter_mode "Interpolation Mode"; t228_QT_dac3_sample_per_cycle "Samples per AXI4-Stream Cycle"; t228_QT_dac3_datapath_mode "Datapath Mode"; t228_QT_dac3_mixer_type "Mixer Type"; t228_QT_dac3_mixer_mode "Mixer Mode"; t228_QT_dac3_nco_freq "NCO Frequency (GHz)"; t228_QT_dac3_nco_phase "NCO Phase"; t228_QT_dac3_coarse_freq "Frequency"; t228_QT_dac3_nyquist_zone "Nyquist Zone"; t228_QT_dac3_decode_mode "Decoder Mode"; t228_DT_dac0_enable "Enable DAC"; t228_DT_dac0_analog_output "Analog Output Data"; t228_DT_dac0_inter_mode "Interpolation Mode"; t228_DT_dac0_sample_per_cycle "Samples per AXI4-Stream Cycle"; t228_DT_dac0_mixer_type "Mixer Type"; t228_DT_dac0_mixer_mode "Mixer Mode"; t228_DT_dac0_nco_freq "NCO Frequency (GHz)"; t228_DT_dac0_nco_phase "NCO Phase"; t228_DT_dac0_coarse_freq "Frequency"; t228_DT_dac0_nyquist_zone "Nyquist Zone"; t228_DT_dac0_decode_mode "Decoder Mode"; t228_DT_dac1_enable "Enable DAC"; t228_DT_dac1_analog_output "Analog Output Data"; t228_DT_dac1_inter_mode "Interpolation Mode"; t228_DT_dac1_sample_per_cycle "Samples per AXI4-Stream Cycle"; t228_DT_dac1_mixer_type "Mixer Type"; t228_DT_dac1_mixer_mode "Mixer Mode"; t228_DT_dac1_nco_freq "NCO Frequency (GHz)"; t228_DT_dac1_nco_phase "NCO Phase"; t228_DT_dac1_coarse_freq "Frequency"; t228_DT_dac1_nyquist_zone "Nyquist Zone"; t228_DT_dac1_decode_mode "Decoder Mode"; Tile229_enable "Enable Tile"; t229_enable_mts "Enable Multi-Tile Sync"; t229_sample_rate "Sampling Rate (Msps)"; t229_clk_out "Clock Out (MHz)"; t229_enable_pll "Enable Tile PLLs"; t229_ref_clk "Reference Clock (MHz)"; t229_axi_stream_clk "Required AXI4-Stream Clock (MHz)"; t229_output_power "Output Power"; t229_QT_dac0_enable "Enable DAC"; t229_QT_dac0_analog_output "Analog Output Data"; t229_QT_dac0_inter_mode "Interpolation Mode"; t229_QT_dac0_sample_per_cycle "Samples per AXI4-Stream Cycle"; t229_QT_dac0_datapath_mode "Datapath Mode"; t229_QT_dac0_mixer_type "Mixer Type"; t229_QT_dac0_mixer_mode "Mixer Mode"; t229_QT_dac0_nco_freq "NCO Frequency (GHz)"; t229_QT_dac0_nco_phase "NCO Phase"; t229_QT_dac0_coarse_freq "Frequency"; t229_QT_dac0_nyquist_zone "Nyquist Zone"; t229_QT_dac0_decode_mode "Decoder Mode"; t229_QT_dac1_enable "Enable DAC"; t229_QT_dac1_analog_output "Analog Output Data"; t229_QT_dac1_inter_mode "Interpolation Mode"; t229_QT_dac1_sample_per_cycle "Samples per AXI4-Stream Cycle"; t229_QT_dac1_datapath_mode "Datapath Mode"; t229_QT_dac1_mixer_type "Mixer Type"; t229_QT_dac1_mixer_mode "Mixer Mode"; t229_QT_dac1_nco_freq "NCO Frequency (GHz)"; t229_QT_dac1_nco_phase "NCO Phase"; t229_QT_dac1_coarse_freq "Frequency"; t229_QT_dac1_nyquist_zone "Nyquist Zone"; t229_QT_dac1_decode_mode "Decoder Mode"; t229_QT_dac2_enable "Enable DAC"; t229_QT_dac2_analog_output "Analog Output Data"; t229_QT_dac2_inter_mode "Interpolation Mode"; t229_QT_dac2_sample_per_cycle "Samples per AXI4-Stream Cycle"; t229_QT_dac2_datapath_mode "Datapath Mode"; t229_QT_dac2_mixer_type "Mixer Type"; t229_QT_dac2_mixer_mode "Mixer Mode"; t229_QT_dac2_nco_freq "NCO Frequency (GHz)"; t229_QT_dac2_nco_phase "NCO Phase"; t229_QT_dac2_coarse_freq "Frequency"; t229_QT_dac2_nyquist_zone "Nyquist Zone"; t229_QT_dac2_decode_mode "Decoder Mode"; t229_QT_dac3_enable "Enable DAC"; t229_QT_dac3_analog_output "Analog Output Data"; t229_QT_dac3_inter_mode "Interpolation Mode"; t229_QT_dac3_sample_per_cycle "Samples per AXI4-Stream Cycle"; t229_QT_dac3_datapath_mode "Datapath Mode"; t229_QT_dac3_mixer_type "Mixer Type"; t229_QT_dac3_mixer_mode "Mixer Mode"; t229_QT_dac3_nco_freq "NCO Frequency (GHz)"; t229_QT_dac3_nco_phase "NCO Phase"; t229_QT_dac3_coarse_freq "Frequency"; t229_QT_dac3_nyquist_zone "Nyquist Zone"; t229_QT_dac3_decode_mode "Decoder Mode"; t229_DT_dac0_enable "Enable DAC"; t229_DT_dac0_analog_output "Analog Output Data"; t229_DT_dac0_inter_mode "Interpolation Mode"; t229_DT_dac0_sample_per_cycle "Samples per AXI4-Stream Cycle"; t229_DT_dac0_mixer_type "Mixer Type"; t229_DT_dac0_mixer_mode "Mixer Mode"; t229_DT_dac0_nco_freq "NCO Frequency (GHz)"; t229_DT_dac0_nco_phase "NCO Phase"; t229_DT_dac0_coarse_freq "Frequency"; t229_DT_dac0_nyquist_zone "Nyquist Zone"; t229_DT_dac0_decode_mode "Decoder Mode"; t229_DT_dac1_enable "Enable DAC"; t229_DT_dac1_analog_output "Analog Output Data"; t229_DT_dac1_inter_mode "Interpolation Mode"; t229_DT_dac1_sample_per_cycle "Samples per AXI4-Stream Cycle"; t229_DT_dac1_mixer_type "Mixer Type"; t229_DT_dac1_mixer_mode "Mixer Mode"; t229_DT_dac1_nco_freq "NCO Frequency (GHz)"; t229_DT_dac1_nco_phase "NCO Phase"; t229_DT_dac1_coarse_freq "Frequency"; t229_DT_dac1_nyquist_zone "Nyquist Zone"; t229_DT_dac1_decode_mode "Decoder Mode"; Tile230_enable "Enable Tile"; t230_enable_mts "Enable Multi-Tile Sync"; t230_sample_rate "Sampling Rate (Msps)"; t230_clk_out "Clock Out (MHz)"; t230_enable_pll "Enable Tile PLLs"; t230_ref_clk "Reference Clock (MHz)"; t230_axi_stream_clk "Required AXI4-Stream Clock (MHz)"; t230_output_power "Output Power"; t230_QT_dac0_enable "Enable DAC"; t230_QT_dac0_analog_output "Analog Output Data"; t230_QT_dac0_inter_mode "Interpolation Mode"; t230_QT_dac0_sample_per_cycle "Samples per AXI4-Stream Cycle"; t230_QT_dac0_datapath_mode "Datapath Mode"; t230_QT_dac0_mixer_type "Mixer Type"; t230_QT_dac0_mixer_mode "Mixer Mode"; t230_QT_dac0_nco_freq "NCO Frequency (GHz)"; t230_QT_dac0_nco_phase "NCO Phase"; t230_QT_dac0_coarse_freq "Frequency"; t230_QT_dac0_nyquist_zone "Nyquist Zone"; t230_QT_dac0_decode_mode "Decoder Mode"; t230_QT_dac1_enable "Enable DAC"; t230_QT_dac1_analog_output "Analog Output Data"; t230_QT_dac1_inter_mode "Interpolation Mode"; t230_QT_dac1_sample_per_cycle "Samples per AXI4-Stream Cycle"; t230_QT_dac1_datapath_mode "Datapath Mode"; t230_QT_dac1_mixer_type "Mixer Type"; t230_QT_dac1_mixer_mode "Mixer Mode"; t230_QT_dac1_nco_freq "NCO Frequency (GHz)"; t230_QT_dac1_nco_phase "NCO Phase"; t230_QT_dac1_coarse_freq "Frequency"; t230_QT_dac1_nyquist_zone "Nyquist Zone"; t230_QT_dac1_decode_mode "Decoder Mode"; t230_QT_dac2_enable "Enable DAC"; t230_QT_dac2_analog_output "Analog Output Data"; t230_QT_dac2_inter_mode "Interpolation Mode"; t230_QT_dac2_sample_per_cycle "Samples per AXI4-Stream Cycle"; t230_QT_dac2_datapath_mode "Datapath Mode"; t230_QT_dac2_mixer_type "Mixer Type"; t230_QT_dac2_mixer_mode "Mixer Mode"; t230_QT_dac2_nco_freq "NCO Frequency (GHz)"; t230_QT_dac2_nco_phase "NCO Phase"; t230_QT_dac2_coarse_freq "Frequency"; t230_QT_dac2_nyquist_zone "Nyquist Zone"; t230_QT_dac2_decode_mode "Decoder Mode"; t230_QT_dac3_enable "Enable DAC"; t230_QT_dac3_analog_output "Analog Output Data"; t230_QT_dac3_inter_mode "Interpolation Mode"; t230_QT_dac3_sample_per_cycle "Samples per AXI4-Stream Cycle"; t230_QT_dac3_datapath_mode "Datapath Mode"; t230_QT_dac3_mixer_type "Mixer Type"; t230_QT_dac3_mixer_mode "Mixer Mode"; t230_QT_dac3_nco_freq "NCO Frequency (GHz)"; t230_QT_dac3_nco_phase "NCO Phase"; t230_QT_dac3_coarse_freq "Frequency"; t230_QT_dac3_nyquist_zone "Nyquist Zone"; t230_QT_dac3_decode_mode "Decoder Mode"; t230_DT_dac0_enable "Enable DAC"; t230_DT_dac0_analog_output "Analog Output Data"; t230_DT_dac0_inter_mode "Interpolation Mode"; t230_DT_dac0_sample_per_cycle "Samples per AXI4-Stream Cycle"; t230_DT_dac0_mixer_type "Mixer Type"; t230_DT_dac0_mixer_mode "Mixer Mode"; t230_DT_dac0_nco_freq "NCO Frequency (GHz)"; t230_DT_dac0_nco_phase "NCO Phase"; t230_DT_dac0_coarse_freq "Frequency"; t230_DT_dac0_nyquist_zone "Nyquist Zone"; t230_DT_dac0_decode_mode "Decoder Mode"; t230_DT_dac1_enable "Enable DAC"; t230_DT_dac1_analog_output "Analog Output Data"; t230_DT_dac1_inter_mode "Interpolation Mode"; t230_DT_dac1_sample_per_cycle "Samples per AXI4-Stream Cycle"; t230_DT_dac1_mixer_type "Mixer Type"; t230_DT_dac1_mixer_mode "Mixer Mode"; t230_DT_dac1_nco_freq "NCO Frequency (GHz)"; t230_DT_dac1_nco_phase "NCO Phase"; t230_DT_dac1_coarse_freq "Frequency"; t230_DT_dac1_nyquist_zone "Nyquist Zone"; t230_DT_dac1_decode_mode "Decoder Mode"; Tile231_enable "Enable Tile"; t231_enable_mts "Enable Multi-Tile Sync"; t231_sample_rate "Sampling Rate (Msps)"; t231_clk_out "Clock Out (MHz)"; t231_enable_pll "Enable Tile PLLs"; t231_ref_clk "Reference Clock (MHz)"; t231_axi_stream_clk "Required AXI4-Stream Clock (MHz)"; t231_output_power "Output Power"; t231_QT_dac0_enable "Enable DAC"; t231_QT_dac0_analog_output "Analog Output Data"; t231_QT_dac0_inter_mode "Interpolation Mode"; t231_QT_dac0_sample_per_cycle "Samples per AXI4-Stream Cycle"; t231_QT_dac0_datapath_mode "Datapath Mode"; t231_QT_dac0_mixer_type "Mixer Type"; t231_QT_dac0_mixer_mode "Mixer Mode"; t231_QT_dac0_nco_freq "NCO Frequency (GHz)"; t231_QT_dac0_nco_phase "NCO Phase"; t231_QT_dac0_coarse_freq "Frequency"; t231_QT_dac0_nyquist_zone "Nyquist Zone"; t231_QT_dac0_decode_mode "Decoder Mode"; t231_QT_dac1_enable "Enable DAC"; t231_QT_dac1_analog_output "Analog Output Data"; t231_QT_dac1_inter_mode "Interpolation Mode"; t231_QT_dac1_sample_per_cycle "Samples per AXI4-Stream Cycle"; t231_QT_dac1_datapath_mode "Datapath Mode"; t231_QT_dac1_mixer_type "Mixer Type"; t231_QT_dac1_mixer_mode "Mixer Mode"; t231_QT_dac1_nco_freq "NCO Frequency (GHz)"; t231_QT_dac1_nco_phase "NCO Phase"; t231_QT_dac1_coarse_freq "Frequency"; t231_QT_dac1_nyquist_zone "Nyquist Zone"; t231_QT_dac1_decode_mode "Decoder Mode"; t231_QT_dac2_enable "Enable DAC"; t231_QT_dac2_analog_output "Analog Output Data"; t231_QT_dac2_inter_mode "Interpolation Mode"; t231_QT_dac2_sample_per_cycle "Samples per AXI4-Stream Cycle"; t231_QT_dac2_datapath_mode "Datapath Mode"; t231_QT_dac2_mixer_type "Mixer Type"; t231_QT_dac2_mixer_mode "Mixer Mode"; t231_QT_dac2_nco_freq "NCO Frequency (GHz)"; t231_QT_dac2_nco_phase "NCO Phase"; t231_QT_dac2_coarse_freq "Frequency"; t231_QT_dac2_nyquist_zone "Nyquist Zone"; t231_QT_dac2_decode_mode "Decoder Mode"; t231_QT_dac3_enable "Enable DAC"; t231_QT_dac3_analog_output "Analog Output Data"; t231_QT_dac3_inter_mode "Interpolation Mode"; t231_QT_dac3_sample_per_cycle "Samples per AXI4-Stream Cycle"; t231_QT_dac3_datapath_mode "Datapath Mode"; t231_QT_dac3_mixer_type "Mixer Type"; t231_QT_dac3_mixer_mode "Mixer Mode"; t231_QT_dac3_nco_freq "NCO Frequency (GHz)"; t231_QT_dac3_nco_phase "NCO Phase"; t231_QT_dac3_coarse_freq "Frequency"; t231_QT_dac3_nyquist_zone "Nyquist Zone"; t231_QT_dac3_decode_mode "Decoder Mode"; t231_DT_dac0_enable "Enable DAC"; t231_DT_dac0_analog_output "Analog Output Data"; t231_DT_dac0_inter_mode "Interpolation Mode"; t231_DT_dac0_sample_per_cycle "Samples per AXI4-Stream Cycle"; t231_DT_dac0_mixer_type "Mixer Type"; t231_DT_dac0_mixer_mode "Mixer Mode"; t231_DT_dac0_nco_freq "NCO Frequency (GHz)"; t231_DT_dac0_nco_phase "NCO Phase"; t231_DT_dac0_coarse_freq "Frequency"; t231_DT_dac0_nyquist_zone "Nyquist Zone"; t231_DT_dac0_decode_mode "Decoder Mode"; t231_DT_dac1_enable "Enable DAC"; t231_DT_dac1_analog_output "Analog Output Data"; t231_DT_dac1_inter_mode "Interpolation Mode"; t231_DT_dac1_sample_per_cycle "Samples per AXI4-Stream Cycle"; t231_DT_dac1_mixer_type "Mixer Type"; t231_DT_dac1_mixer_mode "Mixer Mode"; t231_DT_dac1_nco_freq "NCO Frequency (GHz)"; t231_DT_dac1_nco_phase "NCO Phase"; t231_DT_dac1_coarse_freq "Frequency"; t231_DT_dac1_nyquist_zone "Nyquist Zone"; t231_DT_dac1_decode_mode "Decoder Mode"; t224_has_adc_clk "Has Clock"; t224_adc_clk_src "Clock Source Tile"; t224_clk_dist "Distribute Clock"; t225_has_adc_clk "Has Clock"; t225_adc_clk_src "Clock Source Tile"; t225_clk_dist "Distribute Clock"; t226_has_adc_clk "Has Clock"; t226_adc_clk_src "Clock Source Tile"; t226_clk_dist "Distribute Clock"; t227_has_adc_clk "Has Clock"; t227_adc_clk_src "Clock Source Tile"; t227_clk_dist "Distribute Clock"; t228_has_dac_clk "Has Clock"; t228_dac_clk_src "Clock Source Tile"; t228_clk_dist "Distribute Clock"; t229_has_dac_clk "Has Clock"; t229_dac_clk_src "Clock Source Tile"; t229_clk_dist "Distribute Clock"; t230_has_dac_clk "Has Clock"; t230_dac_clk_src "Clock Source Tile"; t230_clk_dist "Distribute Clock"; t231_has_dac_clk "Has Clock"; t231_dac_clk_src "Clock Source Tile"; t231_clk_dist "Distribute Clock"
      mask help: CASPER RFDC
      mask init:
      | if chk_param(gcb,'runinit','1')
      |     if chk_param(gcb,'forceredraw','0')
      |         rfdc_mask(gcb,0);
      |     else
      |         rfdc_mask(gcb,1);
      |         set_param(gcb,'forceredraw','0')
      |     end
      |     if chk_param(gcb,'maskopening','1')
      |         set_param(gcb,'runinit','0')
      |     end
      | end
      mask Help: eval('xlWeb([getenv(''MLIB_ROOT''), ''\doc\html\adc_zcu111\adc_zcu111.html''])')
      mask Callback maskopening:
      | %assignin('base','mask_opening',1)
      | %assignin('base','run_init',1)
      | set_param(gcb,'maskopening','1')
      mask Callback runinit: set_param(gcb,'runinit','1')
      mask Callback Tile224_enable: enable_mts_opt(gcb);
      mask Callback t224_sample_rate: update_rfdc_clocking(gcb,224);
      mask TypeOptions t224_clk_out: 100 | 50 | 25 | 12.5
      mask Callback t224_enable_pll:
      | %update_rfdc_clocking(gcb);
      | update_pll(gcb,224);
      mask TypeOptions t224_ref_clk: 738.462 | 685.714 | 640 | 600 | 564.706 | 533.333 | 505.263 | 480 | 457.143 | 436.364 | 417.391 | 400 | 384 | 369.231 | 355.556 | 342.857 | 331.034 | 320 | 309.677 | 300 | 290.909 | 282.353 | 274.286 | 266.667 | 259.459 | 252.632 | 246.154 | 240 | 234.146 | 228.571 | 223.256 | 218.182 | 213.333 | 208.696 | 204.255 | 200 | 195.918 | 192 | 188.235 | 184.615 | 181.132 | 177.778 | 174.545 | 171.429 | 168.421 | 165.517 | 162.712 | 160 | 157.377 | 154.839 | 152.381 | 150 | 147.692 | 145.455 | 143.284 | 141.176 | 139.13 | 137.143 | 135.211 | 133.333 | 131.507 | 129.73 | 128 | 126.316 | 124.675 | 123.077 | 121.519 | 120 | 118.519 | 117.073 | 115.663 | 114.286 | 112.941 | 111.628 | 110.345 | 109.091 | 107.865 | 106.667 | 105.495 | 104.348 | 103.226
      mask Callback t224_QT_adc0_enable: enable_adc_opt(gcb,224,0,'QT');
      mask TypeOptions t224_QT_adc0_digital_output: Real | I/Q
      mask Callback t224_QT_adc0_digital_output:
      | validate_digital_data(gcb,224,0,'QT');
      | update_axis_clk(gcb,224);
      mask TypeOptions t224_QT_adc0_dec_mode: 1x | 2x | 3x | 4x | 5x | 6x | 8x | 10x | 12x | 16x | 20x | 24x | 40x
      mask Callback t224_QT_adc0_dec_mode:
      | % if I/Q output mode, need to copy interp factor before updating axis clk
      | % note only the even slice for the tile makes this check
      | if chk_param(gcb, 't224_QT_adc0_mixer_mode', 'I/Q -> I/Q')
      |   dec_mode = get_param(gcb, 't224_QT_adc0_dec_mode');
      |   set_param(gcb, 't224_QT_adc1_dec_mode', dec_mode);
      | end
      | 
      | update_axis_clk(gcb,224);
      mask TypeOptions t224_QT_adc0_sample_per_cycle: 4 | 5 | 6 | 7 | 8 | 9 | 10 | 11 | 12
      mask Callback t224_QT_adc0_sample_per_cycle:
      | % if I/Q output mode, need to copy samples per clk before updating axis clk
      | % note only the even slice for the tile makes this check
      | if chk_param(gcb, 't224_QT_adc0_mixer_mode', 'I/Q -> I/Q')
      |   spc = get_param(gcb, 't224_QT_adc0_sample_per_cycle');
      |   set_param(gcb, 't224_QT_adc1_sample_per_cycle', spc);
      | end
      | update_axis_clk_label(gcb,224);
      mask TypeOptions t224_QT_adc0_mixer_type: Bypassed
      mask Callback t224_QT_adc0_mixer_type: mixertype_callback(gcb,224,0,'QT');
      mask TypeOptions t224_QT_adc0_mixer_mode: Real -> Real
      mask Callback t224_QT_adc0_mixer_mode: mixer_callback(gcb,224,0,'QT');
      mask TypeOptions t224_QT_adc0_coarse_freq: 0
      mask TypeOptions t224_QT_adc0_nyquist_zone: Zone 1 | Zone 2
      mask TypeOptions t224_QT_adc0_cal_mode: Mode 1 | Mode 2
      mask Callback t224_QT_adc1_enable: enable_adc_opt(gcb,224,1,'QT');
      mask TypeOptions t224_QT_adc1_digital_output: Real | I/Q
      mask Callback t224_QT_adc1_digital_output:
      | validate_digital_data(gcb,224,1,'QT');
      | update_axis_clk(gcb,224);
      mask TypeOptions t224_QT_adc1_dec_mode: 1x | 2x | 3x | 4x | 5x | 6x | 8x | 10x | 12x | 16x | 20x | 24x | 40x
      mask Callback t224_QT_adc1_dec_mode: update_axis_clk(gcb,224);
      mask TypeOptions t224_QT_adc1_sample_per_cycle: 4 | 5 | 6 | 7 | 8 | 9 | 10 | 11 | 12
      mask Callback t224_QT_adc1_sample_per_cycle: update_axis_clk_label(gcb,224);
      mask TypeOptions t224_QT_adc1_mixer_type: Bypassed
      mask Callback t224_QT_adc1_mixer_type: mixertype_callback(gcb,224,1,'QT');
      mask TypeOptions t224_QT_adc1_mixer_mode: Real -> Real
      mask Callback t224_QT_adc1_mixer_mode: mixer_callback(gcb,224,1,'QT')
      mask TypeOptions t224_QT_adc1_coarse_freq: 0
      mask TypeOptions t224_QT_adc1_nyquist_zone: Zone 1 | Zone 2
      mask TypeOptions t224_QT_adc1_cal_mode: Mode 1 | Mode 2
      mask Callback t224_QT_adc2_enable: enable_adc_opt(gcb,224,2,'QT');
      mask TypeOptions t224_QT_adc2_digital_output: Real | I/Q
      mask Callback t224_QT_adc2_digital_output:
      | validate_digital_data(gcb,224,2,'QT');
      | update_axis_clk(gcb,224);
      mask TypeOptions t224_QT_adc2_dec_mode: 1x | 2x | 3x | 4x | 5x | 6x | 8x | 10x | 12x | 16x | 20x | 24x | 40x
      mask Callback t224_QT_adc2_dec_mode:
      | % if I/Q output mode, need to copy interp factor before updating axis clk
      | % note only the even slice for the tile makes this check
      | if chk_param(gcb, 't224_QT_adc2_mixer_mode', 'I/Q -> I/Q')
      |   dec_mode = get_param(gcb, 't224_QT_adc2_dec_mode');
      |   set_param(gcb, 't224_QT_adc3_dec_mode', dec_mode);
      | end
      | update_axis_clk(gcb,224);
      mask TypeOptions t224_QT_adc2_sample_per_cycle: 4 | 5 | 6 | 7 | 8 | 9 | 10 | 11 | 12
      mask Callback t224_QT_adc2_sample_per_cycle:
      | % if I/Q output mode, need to copy samples per clk before updating axis clk
      | % note only the even slice for the tile makes this check
      | if chk_param(gcb, 't224_QT_adc2_mixer_mode', 'I/Q -> I/Q')
      |   spc = get_param(gcb, 't224_QT_adc2_sample_per_cycle');
      |   set_param(gcb, 't224_QT_adc3_sample_per_cycle', spc);
      | end
      | update_axis_clk_label(gcb,224);
      mask TypeOptions t224_QT_adc2_mixer_type: Bypassed
      mask Callback t224_QT_adc2_mixer_type: mixertype_callback(gcb,224,2,'QT');
      mask TypeOptions t224_QT_adc2_mixer_mode: Real -> Real
      mask Callback t224_QT_adc2_mixer_mode: mixer_callback(gcb,224,2,'QT')
      mask TypeOptions t224_QT_adc2_coarse_freq: 0
      mask TypeOptions t224_QT_adc2_nyquist_zone: Zone 1 | Zone 2
      mask TypeOptions t224_QT_adc2_cal_mode: Mode 1 | Mode 2
